simulink model "r2_b8a4x128f_4gbe"  (R2012b)
(part 4 of 182)

      |     current_names = textscan(strtrim(strrep(strrep(get_param(blk, 'names'), ']', ''), '[', '')), '%s');
      |     current_names = current_names{1};
      |     numios = length(current_names);
      |     if length(current_widths) ~= numios,
      |         error('%d field names specified, but %d widths?', numios, length(current_widths));
      |     end
      | end
      | total_width = 0;
      | for ctr = 1 : length(current_widths),
      |     total_width = total_width + current_widths(ctr);
      | end
      | if total_width > 32,
      |     error('Total width must be 32 or less, set to %d.', total_width);
      | end
      mask Callback arith_types:
      | blk = gcb;
      | mode = get_param(blk, 'mode');
      | current_types = eval(get_param(blk, 'arith_types'));
      | numios = length(current_types);
      | if (strcmp(mode, 'one value') || strcmp(mode, 'fields of equal size')) && (length(current_types) > 1),
      |     error('Only one type may be specified for this mode.');
      | elseif strcmp(mode, 'fields of arbitrary size')
      |     current_names = textscan(strtrim(strrep(strrep(get_param(blk, 'names'), ']', ''), '[', '')), '%s');
      |     current_names = current_names{1};
      |     numios = length(current_names);
      |     if length(current_types) ~= numios,
      |         error('%d field names specified, but %d types?', numios, length(current_types));
      |     end
      | end
      | problem = 0;
      | for ctr = 1 : numios,
      |     t = current_types(ctr);
      |     if (t < 0) || (t > 2),
      |         problem = t;
      |         ctr = numios + 1;
      |     end
      | end
      | if problem ~= 0,
      |     error('Type cannot be %i, must be 0, 1 or 2.', problem);
      | end
      mask Callback bin_pts:
      | blk = gcb;
      | mode = get_param(blk, 'mode');
      | current_bins = eval(get_param(blk, 'bin_pts'));
      | if (strcmp(mode, 'one value') || strcmp(mode, 'fields of equal size')) && (length(current_bins) > 1),
      |     error('Only one binary pt may be specified for this mode.');
      | elseif strcmp(mode, 'fields of arbitrary size')
      |     current_names = textscan(strtrim(strrep(strrep(get_param(blk, 'names'), ']', ''), '[', '')), '%s');
      |     current_names = current_names{1};
      |     numios = length(current_names);
      |     if length(current_bins) ~= numios,
      |         error('%d field names specified, but %d binary pts?', numios, length(current_bins));
      |     end
      | end
  status1 : Subsystem  Tag=xps:sw_reg  AncestorBlock=xps_library/software register  mask(swreg){mode=fields of equal size, io_dir=To Processor, io_delay=2, sample_period=1, names=[gbe_down rx_dest_err feng_rx_err fft_err feng_qdr_err feng_chk_err adc_over noise_diode_en vacc_err rx_bad_pkt rx_bad_frame tx_over xeng_bad_dat pack_err rxing_data txing_data flushed], bitwidths=1, arith_types=2, bin_pts=0, sim_port=off, show_format=off}
      mask prompts: io_dir "I/O direction"; io_delay "I/O delay"; sample_period "Sample period"; names "Names [msb ... lsb]:"; bitwidths "Bitwidth:"; arith_types "Type (ufix=0, fix=1, bool=2):"; bin_pts "Binary pt:"; sim_port "Provide sim input/output?"; show_format "Print format string?"
      mask init:
      | swreg_init(gcb)
      settings: AttributesFormatString=17 outputs
      mask TypeOptions mode: one value | fields of equal size | fields of arbitrary size
      mask Callback mode: swreg_cb(gcb);
      mask TypeOptions io_dir: To Processor | From Processor
      mask Callback io_dir:
      | mask_enables = get_param(gcb, 'MaskEnables');
      | mask_names = get_param(gcb, 'MaskNames');
      | if strcmp(get_param(gcb, 'io_dir'), 'To Processor'),
      |     mask_enables{ismember(mask_names, 'sample_period')} = 'off';
      | else
      |     mask_enables{ismember(mask_names, 'sample_period')} = 'on';
      | end
      | set_param(gcb, 'MaskEnables', mask_enables);
      mask Callback bitwidths:
      | blk = gcb;
      | mode = get_param(blk, 'mode');
      | current_widths = eval(get_param(blk, 'bitwidths'));
      | if (strcmp(mode, 'one value') || strcmp(mode, 'fields of equal size')) && (length(current_widths) > 1),
      |     error('Only one width may be specified for this mode.');
      | elseif strcmp(mode, 'fields of arbitrary size')
      |     current_names = textscan(strtrim(strrep(strrep(get_param(blk, 'names'), ']', ''), '[', '')), '%s');
      |     current_names = current_names{1};
      |     numios = length(current_names);
      |     if length(current_widths) ~= numios,
      |         error('%d field names specified, but %d widths?', numios, length(current_widths));
      |     end
      | end
      | total_width = 0;
      | for ctr = 1 : length(current_widths),
      |     total_width = total_width + current_widths(ctr);
      | end
      | if total_width > 32,
      |     error('Total width must be 32 or less, set to %d.', total_width);
      | end
      mask Callback arith_types:
      | blk = gcb;
      | mode = get_param(blk, 'mode');
      | current_types = eval(get_param(blk, 'arith_types'));
      | numios = length(current_types);
      | if (strcmp(mode, 'one value') || strcmp(mode, 'fields of equal size')) && (length(current_types) > 1),
      |     error('Only one type may be specified for this mode.');
      | elseif strcmp(mode, 'fields of arbitrary size')
      |     current_names = textscan(strtrim(strrep(strrep(get_param(blk, 'names'), ']', ''), '[', '')), '%s');
      |     current_names = current_names{1};
      |     numios = length(current_names);
      |     if length(current_types) ~= numios,
      |         error('%d field names specified, but %d types?', numios, length(current_types));
      |     end
      | end
      | problem = 0;
      | for ctr = 1 : numios,
      |     t = current_types(ctr);
      |     if (t < 0) || (t > 2),
      |         problem = t;
      |         ctr = numios + 1;
      |     end
      | end
      | if problem ~= 0,
      |     error('Type cannot be %i, must be 0, 1 or 2.', problem);
      | end
      mask Callback bin_pts:
      | blk = gcb;
      | mode = get_param(blk, 'mode');
      | current_bins = eval(get_param(blk, 'bin_pts'));
      | if (strcmp(mode, 'one value') || strcmp(mode, 'fields of equal size')) && (length(current_bins) > 1),
      |     error('Only one binary pt may be specified for this mode.');
      | elseif strcmp(mode, 'fields of arbitrary size')
      |     current_names = textscan(strtrim(strrep(strrep(get_param(blk, 'names'), ']', ''), '[', '')), '%s');
      |     current_names = current_names{1};
      |     numios = length(current_names);
      |     if length(current_bins) ~= numios,
      |         error('%d field names specified, but %d binary pts?', numios, length(current_bins));
      |     end
      | end
  status2 : Subsystem  Tag=xps:sw_reg  AncestorBlock=xps_library/software register  mask(swreg){mode=fields of equal size, io_dir=To Processor, io_delay=2, sample_period=1, names=[gbe_down rx_dest_err feng_rx_err fft_err feng_qdr_err feng_chk_err adc_over noise_diode_en vacc_err rx_bad_pkt rx_bad_frame tx_over xeng_bad_dat pack_err rxing_data txing_data flushed], bitwidths=1, arith_types=2, bin_pts=0, sim_port=off, show_format=off}
      mask prompts: io_dir "I/O direction"; io_delay "I/O delay"; sample_period "Sample period"; names "Names [msb ... lsb]:"; bitwidths "Bitwidth:"; arith_types "Type (ufix=0, fix=1, bool=2):"; bin_pts "Binary pt:"; sim_port "Provide sim input/output?"; show_format "Print format string?"
      mask init:
      | swreg_init(gcb)
      settings: AttributesFormatString=17 outputs
      mask TypeOptions mode: one value | fields of equal size | fields of arbitrary size
      mask Callback mode: swreg_cb(gcb);
      mask TypeOptions io_dir: To Processor | From Processor
      mask Callback io_dir:
      | mask_enables = get_param(gcb, 'MaskEnables');
      | mask_names = get_param(gcb, 'MaskNames');
      | if strcmp(get_param(gcb, 'io_dir'), 'To Processor'),
      |     mask_enables{ismember(mask_names, 'sample_period')} = 'off';
      | else
      |     mask_enables{ismember(mask_names, 'sample_period')} = 'on';
      | end
      | set_param(gcb, 'MaskEnables', mask_enables);
      mask Callback bitwidths:
      | blk = gcb;
      | mode = get_param(blk, 'mode');
      | current_widths = eval(get_param(blk, 'bitwidths'));
      | if (strcmp(mode, 'one value') || strcmp(mode, 'fields of equal size')) && (length(current_widths) > 1),
      |     error('Only one width may be specified for this mode.');
      | elseif strcmp(mode, 'fields of arbitrary size')
      |     current_names = textscan(strtrim(strrep(strrep(get_param(blk, 'names'), ']', ''), '[', '')), '%s');
      |     current_names = current_names{1};
      |     numios = length(current_names);
      |     if length(current_widths) ~= numios,
      |         error('%d field names specified, but %d widths?', numios, length(current_widths));
      |     end
      | end
      | total_width = 0;
      | for ctr = 1 : length(current_widths),
      |     total_width = total_width + current_widths(ctr);
      | end
      | if total_width > 32,
      |     error('Total width must be 32 or less, set to %d.', total_width);
      | end
      mask Callback arith_types:
      | blk = gcb;
      | mode = get_param(blk, 'mode');
      | current_types = eval(get_param(blk, 'arith_types'));
      | numios = length(current_types);
      | if (strcmp(mode, 'one value') || strcmp(mode, 'fields of equal size')) && (length(current_types) > 1),
      |     error('Only one type may be specified for this mode.');
      | elseif strcmp(mode, 'fields of arbitrary size')
      |     current_names = textscan(strtrim(strrep(strrep(get_param(blk, 'names'), ']', ''), '[', '')), '%s');
      |     current_names = current_names{1};
      |     numios = length(current_names);
      |     if length(current_types) ~= numios,
      |         error('%d field names specified, but %d types?', numios, length(current_types));
      |     end
      | end
      | problem = 0;
      | for ctr = 1 : numios,
      |     t = current_types(ctr);
      |     if (t < 0) || (t > 2),
      |         problem = t;
      |         ctr = numios + 1;
      |     end
      | end
      | if problem ~= 0,
      |     error('Type cannot be %i, must be 0, 1 or 2.', problem);
      | end
      mask Callback bin_pts:
      | blk = gcb;
      | mode = get_param(blk, 'mode');
      | current_bins = eval(get_param(blk, 'bin_pts'));
      | if (strcmp(mode, 'one value') || strcmp(mode, 'fields of equal size')) && (length(current_bins) > 1),
      |     error('Only one binary pt may be specified for this mode.');
      | elseif strcmp(mode, 'fields of arbitrary size')
      |     current_names = textscan(strtrim(strrep(strrep(get_param(blk, 'names'), ']', ''), '[', '')), '%s');
      |     current_names = current_names{1};
      |     numios = length(current_names);
      |     if length(current_bins) ~= numios,
      |         error('%d field names specified, but %d binary pts?', numios, length(current_bins));
      |     end
      | end
  status3 : Subsystem  Tag=xps:sw_reg  AncestorBlock=xps_library/software register  mask(swreg){mode=fields of equal size, io_dir=To Processor, io_delay=2, sample_period=1, names=[gbe_down rx_dest_err feng_rx_err fft_err feng_qdr_err feng_chk_err adc_over noise_diode_en vacc_err rx_bad_pkt rx_bad_frame tx_over xeng_bad_dat pack_err rxing_data txing_data flushed], bitwidths=1, arith_types=2, bin_pts=0, sim_port=off, show_format=off}
      mask prompts: io_dir "I/O direction"; io_delay "I/O delay"; sample_period "Sample period"; names "Names [msb ... lsb]:"; bitwidths "Bitwidth:"; arith_types "Type (ufix=0, fix=1, bool=2):"; bin_pts "Binary pt:"; sim_port "Provide sim input/output?"; show_format "Print format string?"
      mask init:
      | swreg_init(gcb)
      settings: AttributesFormatString=17 outputs
      mask TypeOptions mode: one value | fields of equal size | fields of arbitrary size
      mask Callback mode: swreg_cb(gcb);
      mask TypeOptions io_dir: To Processor | From Processor
      mask Callback io_dir:
      | mask_enables = get_param(gcb, 'MaskEnables');
      | mask_names = get_param(gcb, 'MaskNames');
      | if strcmp(get_param(gcb, 'io_dir'), 'To Processor'),
      |     mask_enables{ismember(mask_names, 'sample_period')} = 'off';
      | else
      |     mask_enables{ismember(mask_names, 'sample_period')} = 'on';
      | end
      | set_param(gcb, 'MaskEnables', mask_enables);
      mask Callback bitwidths:
      | blk = gcb;
      | mode = get_param(blk, 'mode');
      | current_widths = eval(get_param(blk, 'bitwidths'));
      | if (strcmp(mode, 'one value') || strcmp(mode, 'fields of equal size')) && (length(current_widths) > 1),
      |     error('Only one width may be specified for this mode.');
      | elseif strcmp(mode, 'fields of arbitrary size')
      |     current_names = textscan(strtrim(strrep(strrep(get_param(blk, 'names'), ']', ''), '[', '')), '%s');
      |     current_names = current_names{1};
      |     numios = length(current_names);
      |     if length(current_widths) ~= numios,
      |         error('%d field names specified, but %d widths?', numios, length(current_widths));
      |     end
      | end
      | total_width = 0;
      | for ctr = 1 : length(current_widths),
      |     total_width = total_width + current_widths(ctr);
      | end
      | if total_width > 32,
      |     error('Total width must be 32 or less, set to %d.', total_width);
      | end
      mask Callback arith_types:
      | blk = gcb;
      | mode = get_param(blk, 'mode');
      | current_types = eval(get_param(blk, 'arith_types'));
      | numios = length(current_types);
      | if (strcmp(mode, 'one value') || strcmp(mode, 'fields of equal size')) && (length(current_types) > 1),
      |     error('Only one type may be specified for this mode.');
      | elseif strcmp(mode, 'fields of arbitrary size')
      |     current_names = textscan(strtrim(strrep(strrep(get_param(blk, 'names'), ']', ''), '[', '')), '%s');
      |     current_names = current_names{1};
      |     numios = length(current_names);
      |     if length(current_types) ~= numios,
      |         error('%d field names specified, but %d types?', numios, length(current_types));
      |     end
      | end
      | problem = 0;
      | for ctr = 1 : numios,
      |     t = current_types(ctr);
      |     if (t < 0) || (t > 2),
      |         problem = t;
      |         ctr = numios + 1;
      |     end
      | end
      | if problem ~= 0,
      |     error('Type cannot be %i, must be 0, 1 or 2.', problem);
      | end
      mask Callback bin_pts:
      | blk = gcb;
      | mode = get_param(blk, 'mode');
      | current_bins = eval(get_param(blk, 'bin_pts'));
      | if (strcmp(mode, 'one value') || strcmp(mode, 'fields of equal size')) && (length(current_bins) > 1),
      |     error('Only one binary pt may be specified for this mode.');
      | elseif strcmp(mode, 'fields of arbitrary size')
      |     current_names = textscan(strtrim(strrep(strrep(get_param(blk, 'names'), ']', ''), '[', '')), '%s');
      |     current_names = current_names{1};
      |     numios = length(current_names);
      |     if length(current_bins) ~= numios,
      |         error('%d field names specified, but %d binary pts?', numios, length(current_bins));
      |     end
      | end
  sys0 : Subsystem  mask{n_bits_channels=fft_stages-1, n_bits_xengs=n_bits_xengs, n_bits_ants=n_ants, n_bits_xengs_per_fpga=2, xeng_id=0}
      mask prompts: n_bits_channels "frequency channels (2^?)"; n_bits_xengs "xengines in system (2^?)"; n_bits_ants "antennas in system (2^?)"; n_bits_xengs_per_fpga "xengs per fpga (2^?)"; xeng_id "xeng offset in this fpga"
      mask Display: text(0.1, 0.5, 'PREPROCESS -> REORDER -> XENG -> VACC -> PACK');
  sys1 : Subsystem  mask{n_bits_channels=fft_stages-1, n_bits_xengs=n_bits_xengs, n_bits_ants=n_ants, n_bits_xengs_per_fpga=2, xeng_id=1}
      mask prompts: n_bits_channels "frequency channels (2^?)"; n_bits_xengs "xengines in system (2^?)"; n_bits_ants "antennas in systems (2^?)"; n_bits_xengs_per_fpga "xengs per fpga (2^?)"; xeng_id "xeng offset in this fpga"
      mask Display: text(0.1, 0.5, 'PREPROCESS -> REORDER -> XENG -> VACC -> PACK');
  sys2 : Subsystem  mask{n_bits_channels=fft_stages-1, n_bits_xengs=n_bits_xengs, n_bits_ants=n_ants, n_bits_xengs_per_fpga=2, xeng_id=2}
      mask prompts: n_bits_channels "frequency channels (2^?)"; n_bits_xengs "xengines in system (2^?)"; n_bits_ants "antennas in systems (2^?)"; n_bits_xengs_per_fpga "xengs per fpga (2^?)"; xeng_id "xeng offset in this fpga"
      mask Display: text(0.1, 0.5, 'PREPROCESS -> REORDER -> XENG -> VACC -> PACK');
  sys3 : Subsystem  mask{n_bits_channels=fft_stages-1, n_bits_xengs=n_bits_xengs, n_bits_ants=n_ants, n_bits_xengs_per_fpga=2, xeng_id=3}
      mask prompts: n_bits_channels "frequency channels (2^?)"; n_bits_xengs "xengines in system (2^?)"; n_bits_ants "antennas in systems (2^?)"; n_bits_xengs_per_fpga "xengs per fpga (2^?)"; xeng_id "xeng offset in this fpga"
      mask Display: text(0.1, 0.5, 'PREPROCESS -> REORDER -> XENG -> VACC -> PACK');
  tvg_control : Subsystem  Tag=xps:sw_reg  AncestorBlock=xps_library/software register  mask(swreg){mode=fields of arbitrary size, io_dir=From Processor, io_delay=0, sample_period=1, names=[xeng vacc], bitwidths=[2 6], arith_types=[0 0], bin_pts=[0 0], sim_port=off, show_format=on}
      mask prompts: io_dir "I/O direction"; io_delay "I/O delay"; sample_period "Sample period"; names "Names [msb ... lsb]:"; bitwidths "Bitwidths [msb ... lsb]:"; arith_types "Types (ufix=0, fix=1, bool=2) [msb ... lsb]:"; bin_pts "Binary pts [msb ... lsb]:"; sim_port "Provide sim input/output?"; show_format "Print format string?"
      mask init:
      | swreg_init(gcb)
      settings: AttributesFormatString=2 inputs:uf2.0,uf6.0,
      mask TypeOptions mode: one value | fields of equal size | fields of arbitrary size
      mask Callback mode: swreg_cb(gcb);
      mask TypeOptions io_dir: To Processor | From Processor
      mask Callback io_dir:
      | mask_enables = get_param(gcb, 'MaskEnables');
      | mask_names = get_param(gcb, 'MaskNames');
      | if strcmp(get_param(gcb, 'io_dir'), 'To Processor'),
      |     mask_enables{ismember(mask_names, 'sample_period')} = 'off';
      | else
      |     mask_enables{ismember(mask_names, 'sample_period')} = 'on';
      | end
      | set_param(gcb, 'MaskEnables', mask_enables);
      mask Callback bitwidths:
      | blk = gcb;
      | mode = get_param(blk, 'mode');
      | current_widths = eval(get_param(blk, 'bitwidths'));
      | if (strcmp(mode, 'one value') || strcmp(mode, 'fields of equal size')) && (length(current_widths) > 1),
      |     error('Only one width may be specified for this mode.');
      | elseif strcmp(mode, 'fields of arbitrary size')
      |     current_names = textscan(strtrim(strrep(strrep(get_param(blk, 'names'), ']', ''), '[', '')), '%s');
      |     current_names = current_names{1};
      |     numios = length(current_names);
      |     if length(current_widths) ~= numios,
      |         error('%d field names specified, but %d widths?', numios, length(current_widths));
      |     end
      | end
      | total_width = 0;
      | for ctr = 1 : length(current_widths),
      |     total_width = total_width + current_widths(ctr);
      | end
      | if total_width > 32,
      |     error('Total width must be 32 or less, set to %d.', total_width);
      | end
      mask Callback arith_types:
      | blk = gcb;
      | mode = get_param(blk, 'mode');
      | current_types = eval(get_param(blk, 'arith_types'));
      | numios = length(current_types);
      | if (strcmp(mode, 'one value') || strcmp(mode, 'fields of equal size')) && (length(current_types) > 1),
      |     error('Only one type may be specified for this mode.');
      | elseif strcmp(mode, 'fields of arbitrary size')
      |     current_names = textscan(strtrim(strrep(strrep(get_param(blk, 'names'), ']', ''), '[', '')), '%s');
      |     current_names = current_names{1};
      |     numios = length(current_names);
      |     if length(current_types) ~= numios,
      |         error('%d field names specified, but %d types?', numios, length(current_types));
      |     end
      | end
      | problem = 0;
      | for ctr = 1 : numios,
      |     t = current_types(ctr);
      |     if (t < 0) || (t > 2),
      |         problem = t;
      |         ctr = numios + 1;
      |     end
      | end
      | if problem ~= 0,
      |     error('Type cannot be %i, must be 0, 1 or 2.', problem);
      | end
      mask Callback bin_pts:
      | blk = gcb;
      | mode = get_param(blk, 'mode');
      | current_bins = eval(get_param(blk, 'bin_pts'));
      | if (strcmp(mode, 'one value') || strcmp(mode, 'fields of equal size')) && (length(current_bins) > 1),
      |     error('Only one binary pt may be specified for this mode.');
      | elseif strcmp(mode, 'fields of arbitrary size')
      |     current_names = textscan(strtrim(strrep(strrep(get_param(blk, 'names'), ']', ''), '[', '')), '%s');
      |     current_names = current_names{1};
      |     numios = length(current_names);
      |     if length(current_bins) ~= numios,
      |         error('%d field names specified, but %d binary pts?', numios, length(current_bins));
      |     end
      | end
  vacc_errors0 : Subsystem  Tag=xps:sw_reg  AncestorBlock=xps_library/software register  mask(swreg){mode=fields of arbitrary size, io_dir=To Processor, io_delay=1, sample_period=1, names=[calfail inputof rst outputof parity], bitwidths=[6 6 6 6 6], arith_types=[0 0 0 0 0], bin_pts=[0 0 0 0 0], sim_port=off, show_format=on}
      mask prompts: io_dir "I/O direction"; io_delay "I/O delay"; sample_period "Sample period"; names "Names [msb ... lsb]:"; bitwidths "Bitwidths [msb ... lsb]:"; arith_types "Types (ufix=0, fix=1, bool=2) [msb ... lsb]:"; bin_pts "Binary pts [msb ... lsb]:"; sim_port "Provide sim input/output?"; show_format "Print format string?"
      mask init:
      | swreg_init(gcb)
      settings: AttributesFormatString=5 outputs:uf6.0,uf6.0,uf6.0,uf6.0,uf6.0,
      mask TypeOptions mode: one value | fields of equal size | fields of arbitrary size
      mask Callback mode: swreg_cb(gcb);
      mask TypeOptions io_dir: To Processor | From Processor
      mask Callback io_dir:
      | mask_enables = get_param(gcb, 'MaskEnables');
      | mask_names = get_param(gcb, 'MaskNames');
      | if strcmp(get_param(gcb, 'io_dir'), 'To Processor'),
      |     mask_enables{ismember(mask_names, 'sample_period')} = 'off';
      | else
      |     mask_enables{ismember(mask_names, 'sample_period')} = 'on';
      | end
      | set_param(gcb, 'MaskEnables', mask_enables);
      mask Callback bitwidths:
      | blk = gcb;
      | mode = get_param(blk, 'mode');
      | current_widths = eval(get_param(blk, 'bitwidths'));
      | if (strcmp(mode, 'one value') || strcmp(mode, 'fields of equal size')) && (length(current_widths) > 1),
      |     error('Only one width may be specified for this mode.');
      | elseif strcmp(mode, 'fields of arbitrary size')
      |     current_names = textscan(strtrim(strrep(strrep(get_param(blk, 'names'), ']', ''), '[', '')), '%s');
      |     current_names = current_names{1};
      |     numios = length(current_names);
      |     if length(current_widths) ~= numios,
      |         error('%d field names specified, but %d widths?', numios, length(current_widths));
      |     end
      | end
      | total_width = 0;
      | for ctr = 1 : length(current_widths),
      |     total_width = total_width + current_widths(ctr);
      | end
      | if total_width > 32,
      |     error('Total width must be 32 or less, set to %d.', total_width);
      | end
      mask Callback arith_types:
      | blk = gcb;
      | mode = get_param(blk, 'mode');
      | current_types = eval(get_param(blk, 'arith_types'));
      | numios = length(current_types);
      | if (strcmp(mode, 'one value') || strcmp(mode, 'fields of equal size')) && (length(current_types) > 1),
      |     error('Only one type may be specified for this mode.');
      | elseif strcmp(mode, 'fields of arbitrary size')
      |     current_names = textscan(strtrim(strrep(strrep(get_param(blk, 'names'), ']', ''), '[', '')), '%s');
      |     current_names = current_names{1};
      |     numios = length(current_names);
      |     if length(current_types) ~= numios,
      |         error('%d field names specified, but %d types?', numios, length(current_types));
      |     end
      | end
      | problem = 0;
      | for ctr = 1 : numios,
      |     t = current_types(ctr);
      |     if (t < 0) || (t > 2),
      |         problem = t;
      |         ctr = numios + 1;
      |     end
      | end
      | if problem ~= 0,
      |     error('Type cannot be %i, must be 0, 1 or 2.', problem);
      | end
      mask Callback bin_pts:
      | blk = gcb;
      | mode = get_param(blk, 'mode');
      | current_bins = eval(get_param(blk, 'bin_pts'));
      | if (strcmp(mode, 'one value') || strcmp(mode, 'fields of equal size')) && (length(current_bins) > 1),
      |     error('Only one binary pt may be specified for this mode.');
      | elseif strcmp(mode, 'fields of arbitrary size')
      |     current_names = textscan(strtrim(strrep(strrep(get_param(blk, 'names'), ']', ''), '[', '')), '%s');
      |     current_names = current_names{1};
      |     numios = length(current_names);
      |     if length(current_bins) ~= numios,
      |         error('%d field names specified, but %d binary pts?', numios, length(current_bins));
      |     end
      | end
  vacc_errors1 : Subsystem  Tag=xps:sw_reg  AncestorBlock=xps_library/software register  mask(swreg){mode=fields of arbitrary size, io_dir=To Processor, io_delay=0, sample_period=1, names=[calfail inputof rst outputof parity], bitwidths=[6 6 6 6 6], arith_types=[0 0 0 0 0], bin_pts=[0 0 0 0 0], sim_port=off, show_format=on}
      mask prompts: io_dir "I/O direction"; io_delay "I/O delay"; sample_period "Sample period"; names "Names [msb ... lsb]:"; bitwidths "Bitwidths [msb ... lsb]:"; arith_types "Types (ufix=0, fix=1, bool=2) [msb ... lsb]:"; bin_pts "Binary pts [msb ... lsb]:"; sim_port "Provide sim input/output?"; show_format "Print format string?"
      mask init:
      | swreg_init(gcb)
      settings: AttributesFormatString=5 outputs:uf6.0,uf6.0,uf6.0,uf6.0,uf6.0,
      mask TypeOptions mode: one value | fields of equal size | fields of arbitrary size
      mask Callback mode: swreg_cb(gcb);
      mask TypeOptions io_dir: To Processor | From Processor
      mask Callback io_dir:
      | mask_enables = get_param(gcb, 'MaskEnables');
      | mask_names = get_param(gcb, 'MaskNames');
      | if strcmp(get_param(gcb, 'io_dir'), 'To Processor'),
      |     mask_enables{ismember(mask_names, 'sample_period')} = 'off';
      | else
      |     mask_enables{ismember(mask_names, 'sample_period')} = 'on';
      | end
      | set_param(gcb, 'MaskEnables', mask_enables);
      mask Callback bitwidths:
      | blk = gcb;
      | mode = get_param(blk, 'mode');
      | current_widths = eval(get_param(blk, 'bitwidths'));
      | if (strcmp(mode, 'one value') || strcmp(mode, 'fields of equal size')) && (length(current_widths) > 1),
      |     error('Only one width may be specified for this mode.');
      | elseif strcmp(mode, 'fields of arbitrary size')
      |     current_names = textscan(strtrim(strrep(strrep(get_param(blk, 'names'), ']', ''), '[', '')), '%s');
      |     current_names = current_names{1};
      |     numios = length(current_names);
      |     if length(current_widths) ~= numios,
      |         error('%d field names specified, but %d widths?', numios, length(current_widths));
      |     end
      | end
      | total_width = 0;
      | for ctr = 1 : length(current_widths),
      |     total_width = total_width + current_widths(ctr);
      | end
      | if total_width > 32,
      |     error('Total width must be 32 or less, set to %d.', total_width);
      | end
      mask Callback arith_types:
      | blk = gcb;
      | mode = get_param(blk, 'mode');
      | current_types = eval(get_param(blk, 'arith_types'));
      | numios = length(current_types);
      | if (strcmp(mode, 'one value') || strcmp(mode, 'fields of equal size')) && (length(current_types) > 1),
      |     error('Only one type may be specified for this mode.');
      | elseif strcmp(mode, 'fields of arbitrary size')
      |     current_names = textscan(strtrim(strrep(strrep(get_param(blk, 'names'), ']', ''), '[', '')), '%s');
      |     current_names = current_names{1};
      |     numios = length(current_names);
      |     if length(current_types) ~= numios,
      |         error('%d field names specified, but %d types?', numios, length(current_types));
      |     end
      | end
      | problem = 0;
      | for ctr = 1 : numios,
      |     t = current_types(ctr);
      |     if (t < 0) || (t > 2),
      |         problem = t;
      |         ctr = numios + 1;
      |     end
      | end
      | if problem ~= 0,
      |     error('Type cannot be %i, must be 0, 1 or 2.', problem);
      | end
      mask Callback bin_pts:
      | blk = gcb;
      | mode = get_param(blk, 'mode');
      | current_bins = eval(get_param(blk, 'bin_pts'));
      | if (strcmp(mode, 'one value') || strcmp(mode, 'fields of equal size')) && (length(current_bins) > 1),
      |     error('Only one binary pt may be specified for this mode.');
      | elseif strcmp(mode, 'fields of arbitrary size')
      |     current_names = textscan(strtrim(strrep(strrep(get_param(blk, 'names'), ']', ''), '[', '')), '%s');
      |     current_names = current_names{1};
      |     numios = length(current_names);
      |     if length(current_bins) ~= numios,
      |         error('%d field names specified, but %d binary pts?', numios, length(current_bins));
      |     end
      | end
  vacc_errors2 : Subsystem  Tag=xps:sw_reg  AncestorBlock=xps_library/software register  mask(swreg){mode=fields of arbitrary size, io_dir=To Processor, io_delay=0, sample_period=1, names=[calfail inputof rst outputof parity], bitwidths=[6 6 6 6 6], arith_types=[0 0 0 0 0], bin_pts=[0 0 0 0 0], sim_port=off, show_format=on}
      mask prompts: io_dir "I/O direction"; io_delay "I/O delay"; sample_period "Sample period"; names "Names [msb ... lsb]:"; bitwidths "Bitwidths [msb ... lsb]:"; arith_types "Types (ufix=0, fix=1, bool=2) [msb ... lsb]:"; bin_pts "Binary pts [msb ... lsb]:"; sim_port "Provide sim input/output?"; show_format "Print format string?"
      mask init:
      | swreg_init(gcb)
      settings: AttributesFormatString=5 outputs:uf6.0,uf6.0,uf6.0,uf6.0,uf6.0,
      mask TypeOptions mode: one value | fields of equal size | fields of arbitrary size
      mask Callback mode: swreg_cb(gcb);
      mask TypeOptions io_dir: To Processor | From Processor
      mask Callback io_dir:
      | mask_enables = get_param(gcb, 'MaskEnables');
      | mask_names = get_param(gcb, 'MaskNames');
      | if strcmp(get_param(gcb, 'io_dir'), 'To Processor'),
      |     mask_enables{ismember(mask_names, 'sample_period')} = 'off';
      | else
      |     mask_enables{ismember(mask_names, 'sample_period')} = 'on';
      | end
      | set_param(gcb, 'MaskEnables', mask_enables);
      mask Callback bitwidths:
      | blk = gcb;
      | mode = get_param(blk, 'mode');
      | current_widths = eval(get_param(blk, 'bitwidths'));
      | if (strcmp(mode, 'one value') || strcmp(mode, 'fields of equal size')) && (length(current_widths) > 1),
      |     error('Only one width may be specified for this mode.');
      | elseif strcmp(mode, 'fields of arbitrary size')
      |     current_names = textscan(strtrim(strrep(strrep(get_param(blk, 'names'), ']', ''), '[', '')), '%s');
      |     current_names = current_names{1};
      |     numios = length(current_names);
      |     if length(current_widths) ~= numios,
      |         error('%d field names specified, but %d widths?', numios, length(current_widths));
      |     end
      | end
      | total_width = 0;
      | for ctr = 1 : length(current_widths),
      |     total_width = total_width + current_widths(ctr);
      | end
      | if total_width > 32,
      |     error('Total width must be 32 or less, set to %d.', total_width);
      | end
      mask Callback arith_types:
      | blk = gcb;
      | mode = get_param(blk, 'mode');
      | current_types = eval(get_param(blk, 'arith_types'));
      | numios = length(current_types);
      | if (strcmp(mode, 'one value') || strcmp(mode, 'fields of equal size')) && (length(current_types) > 1),
      |     error('Only one type may be specified for this mode.');
      | elseif strcmp(mode, 'fields of arbitrary size')
      |     current_names = textscan(strtrim(strrep(strrep(get_param(blk, 'names'), ']', ''), '[', '')), '%s');
      |     current_names = current_names{1};
      |     numios = length(current_names);
      |     if length(current_types) ~= numios,
      |         error('%d field names specified, but %d types?', numios, length(current_types));
      |     end
      | end
      | problem = 0;
      | for ctr = 1 : numios,
      |     t = current_types(ctr);
      |     if (t < 0) || (t > 2),
      |         problem = t;
      |         ctr = numios + 1;
      |     end
      | end
      | if problem ~= 0,
      |     error('Type cannot be %i, must be 0, 1 or 2.', problem);
      | end
      mask Callback bin_pts:
      | blk = gcb;
      | mode = get_param(blk, 'mode');
      | current_bins = eval(get_param(blk, 'bin_pts'));
      | if (strcmp(mode, 'one value') || strcmp(mode, 'fields of equal size')) && (length(current_bins) > 1),
      |     error('Only one binary pt may be specified for this mode.');
      | elseif strcmp(mode, 'fields of arbitrary size')
      |     current_names = textscan(strtrim(strrep(strrep(get_param(blk, 'names'), ']', ''), '[', '')), '%s');
      |     current_names = current_names{1};
      |     numios = length(current_names);
      |     if length(current_bins) ~= numios,
      |         error('%d field names specified, but %d binary pts?', numios, length(current_bins));
      |     end
      | end
  vacc_errors3 : Subsystem  Tag=xps:sw_reg  AncestorBlock=xps_library/software register  mask(swreg){mode=fields of arbitrary size, io_dir=To Processor, io_delay=1, sample_period=1, names=[calfail inputof rst outputof parity], bitwidths=[6 6 6 6 6], arith_types=[0 0 0 0 0], bin_pts=[0 0 0 0 0], sim_port=off, show_format=on}
      mask prompts: io_dir "I/O direction"; io_delay "I/O delay"; sample_period "Sample period"; names "Names [msb ... lsb]:"; bitwidths "Bitwidths [msb ... lsb]:"; arith_types "Types (ufix=0, fix=1, bool=2) [msb ... lsb]:"; bin_pts "Binary pts [msb ... lsb]:"; sim_port "Provide sim input/output?"; show_format "Print format string?"
      mask init:
      | swreg_init(gcb)
      settings: AttributesFormatString=5 outputs:uf6.0,uf6.0,uf6.0,uf6.0,uf6.0,
      mask TypeOptions mode: one value | fields of equal size | fields of arbitrary size
      mask Callback mode: swreg_cb(gcb);
      mask TypeOptions io_dir: To Processor | From Processor
      mask Callback io_dir:
      | mask_enables = get_param(gcb, 'MaskEnables');
      | mask_names = get_param(gcb, 'MaskNames');
      | if strcmp(get_param(gcb, 'io_dir'), 'To Processor'),
      |     mask_enables{ismember(mask_names, 'sample_period')} = 'off';
      | else
      |     mask_enables{ismember(mask_names, 'sample_period')} = 'on';
      | end
      | set_param(gcb, 'MaskEnables', mask_enables);
      mask Callback bitwidths:
      | blk = gcb;
      | mode = get_param(blk, 'mode');
      | current_widths = eval(get_param(blk, 'bitwidths'));
      | if (strcmp(mode, 'one value') || strcmp(mode, 'fields of equal size')) && (length(current_widths) > 1),
      |     error('Only one width may be specified for this mode.');
      | elseif strcmp(mode, 'fields of arbitrary size')
      |     current_names = textscan(strtrim(strrep(strrep(get_param(blk, 'names'), ']', ''), '[', '')), '%s');
      |     current_names = current_names{1};
      |     numios = length(current_names);
      |     if length(current_widths) ~= numios,
      |         error('%d field names specified, but %d widths?', numios, length(current_widths));
      |     end
      | end
      | total_width = 0;
      | for ctr = 1 : length(current_widths),
      |     total_width = total_width + current_widths(ctr);
      | end
      | if total_width > 32,
      |     error('Total width must be 32 or less, set to %d.', total_width);
      | end
      mask Callback arith_types:
      | blk = gcb;
      | mode = get_param(blk, 'mode');
      | current_types = eval(get_param(blk, 'arith_types'));
      | numios = length(current_types);
      | if (strcmp(mode, 'one value') || strcmp(mode, 'fields of equal size')) && (length(current_types) > 1),
      |     error('Only one type may be specified for this mode.');
      | elseif strcmp(mode, 'fields of arbitrary size')
      |     current_names = textscan(strtrim(strrep(strrep(get_param(blk, 'names'), ']', ''), '[', '')), '%s');
      |     current_names = current_names{1};
      |     numios = length(current_names);
      |     if length(current_types) ~= numios,
      |         error('%d field names specified, but %d types?', numios, length(current_types));
      |     end
      | end
      | problem = 0;
      | for ctr = 1 : numios,
      |     t = current_types(ctr);
      |     if (t < 0) || (t > 2),
      |         problem = t;
      |         ctr = numios + 1;
      |     end
      | end
      | if problem ~= 0,
      |     error('Type cannot be %i, must be 0, 1 or 2.', problem);
      | end
      mask Callback bin_pts:
      | blk = gcb;
      | mode = get_param(blk, 'mode');
      | current_bins = eval(get_param(blk, 'bin_pts'));
      | if (strcmp(mode, 'one value') || strcmp(mode, 'fields of equal size')) && (length(current_bins) > 1),
      |     error('Only one binary pt may be specified for this mode.');
      | elseif strcmp(mode, 'fields of arbitrary size')
      |     current_names = textscan(strtrim(strrep(strrep(get_param(blk, 'names'), ']', ''), '[', '')), '%s');
      |     current_names = current_names{1};
      |     numios = length(current_names);
      |     if length(current_bins) ~= numios,
      |         error('%d field names specified, but %d binary pts?', numios, length(current_bins));
      |     end
      | end
  vacc_ld_status0 : Subsystem  Tag=xps:sw_reg  AncestorBlock=xps_library/software register  mask(swreg){mode=fields of equal size, io_dir=To Processor, io_delay=1, sample_period=1, names=[armcnt ldcnt], bitwidths=16, arith_types=0, bin_pts=0, sim_port=off, show_format=on}
      mask prompts: io_dir "I/O direction"; io_delay "I/O delay"; sample_period "Sample period"; names "Names [msb ... lsb]:"; bitwidths "Bitwidth:"; arith_types "Type (ufix=0, fix=1, bool=2):"; bin_pts "Binary pt:"; sim_port "Provide sim input/output?"; show_format "Print format string?"
      mask init:
      | swreg_init(gcb)
      settings: AttributesFormatString=2 outputs:uf16.0,uf16.0,
      mask TypeOptions mode: one value | fields of equal size | fields of arbitrary size
      mask Callback mode: swreg_cb(gcb);
      mask TypeOptions io_dir: To Processor | From Processor
      mask Callback io_dir:
      | mask_enables = get_param(gcb, 'MaskEnables');
      | mask_names = get_param(gcb, 'MaskNames');
      | if strcmp(get_param(gcb, 'io_dir'), 'To Processor'),
      |     mask_enables{ismember(mask_names, 'sample_period')} = 'off';
      | else
      |     mask_enables{ismember(mask_names, 'sample_period')} = 'on';
      | end
      | set_param(gcb, 'MaskEnables', mask_enables);
      mask Callback bitwidths:
      | blk = gcb;
      | mode = get_param(blk, 'mode');
      | current_widths = eval(get_param(blk, 'bitwidths'));
      | if (strcmp(mode, 'one value') || strcmp(mode, 'fields of equal size')) && (length(current_widths) > 1),
      |     error('Only one width may be specified for this mode.');
      | elseif strcmp(mode, 'fields of arbitrary size')
      |     current_names = textscan(strtrim(strrep(strrep(get_param(blk, 'names'), ']', ''), '[', '')), '%s');
      |     current_names = current_names{1};
      |     numios = length(current_names);
      |     if length(current_widths) ~= numios,
      |         error('%d field names specified, but %d widths?', numios, length(current_widths));
      |     end
      | end
      | total_width = 0;
      | for ctr = 1 : length(current_widths),
      |     total_width = total_width + current_widths(ctr);
      | end
      | if total_width > 32,
      |     error('Total width must be 32 or less, set to %d.', total_width);
      | end
      mask Callback arith_types:
      | blk = gcb;
      | mode = get_param(blk, 'mode');
      | current_types = eval(get_param(blk, 'arith_types'));
      | numios = length(current_types);
      | if (strcmp(mode, 'one value') || strcmp(mode, 'fields of equal size')) && (length(current_types) > 1),
      |     error('Only one type may be specified for this mode.');
      | elseif strcmp(mode, 'fields of arbitrary size')
      |     current_names = textscan(strtrim(strrep(strrep(get_param(blk, 'names'), ']', ''), '[', '')), '%s');
      |     current_names = current_names{1};
      |     numios = length(current_names);
      |     if length(current_types) ~= numios,
      |         error('%d field names specified, but %d types?', numios, length(current_types));
      |     end
      | end
      | problem = 0;
      | for ctr = 1 : numios,
      |     t = current_types(ctr);
      |     if (t < 0) || (t > 2),
      |         problem = t;
      |         ctr = numios + 1;
      |     end
      | end
      | if problem ~= 0,
      |     error('Type cannot be %i, must be 0, 1 or 2.', problem);
      | end
      mask Callback bin_pts:
      | blk = gcb;
      | mode = get_param(blk, 'mode');
      | current_bins = eval(get_param(blk, 'bin_pts'));
      | if (strcmp(mode, 'one value') || strcmp(mode, 'fields of equal size')) && (length(current_bins) > 1),
      |     error('Only one binary pt may be specified for this mode.');
      | elseif strcmp(mode, 'fields of arbitrary size')
      |     current_names = textscan(strtrim(strrep(strrep(get_param(blk, 'names'), ']', ''), '[', '')), '%s');
      |     current_names = current_names{1};
      |     numios = length(current_names);
      |     if length(current_bins) ~= numios,
      |         error('%d field names specified, but %d binary pts?', numios, length(current_bins));
      |     end
      | end
  vacc_ld_status1 : Subsystem  Tag=xps:sw_reg  AncestorBlock=xps_library/software register  mask(swreg){mode=fields of equal size, io_dir=To Processor, io_delay=0, sample_period=1, names=[armcnt ldcnt], bitwidths=16, arith_types=0, bin_pts=0, sim_port=off, show_format=on}
      mask prompts: io_dir "I/O direction"; io_delay "I/O delay"; sample_period "Sample period"; names "Names [msb ... lsb]:"; bitwidths "Bitwidth:"; arith_types "Type (ufix=0, fix=1, bool=2):"; bin_pts "Binary pt:"; sim_port "Provide sim input/output?"; show_format "Print format string?"
      mask init:
      | swreg_init(gcb)
      settings: AttributesFormatString=2 outputs:uf16.0,uf16.0,
      mask TypeOptions mode: one value | fields of equal size | fields of arbitrary size
      mask Callback mode: swreg_cb(gcb);
      mask TypeOptions io_dir: To Processor | From Processor
      mask Callback io_dir:
      | mask_enables = get_param(gcb, 'MaskEnables');
      | mask_names = get_param(gcb, 'MaskNames');
      | if strcmp(get_param(gcb, 'io_dir'), 'To Processor'),
      |     mask_enables{ismember(mask_names, 'sample_period')} = 'off';
      | else
      |     mask_enables{ismember(mask_names, 'sample_period')} = 'on';
      | end
      | set_param(gcb, 'MaskEnables', mask_enables);
      mask Callback bitwidths:
      | blk = gcb;
      | mode = get_param(blk, 'mode');
      | current_widths = eval(get_param(blk, 'bitwidths'));
      | if (strcmp(mode, 'one value') || strcmp(mode, 'fields of equal size')) && (length(current_widths) > 1),
      |     error('Only one width may be specified for this mode.');
      | elseif strcmp(mode, 'fields of arbitrary size')
      |     current_names = textscan(strtrim(strrep(strrep(get_param(blk, 'names'), ']', ''), '[', '')), '%s');
      |     current_names = current_names{1};
      |     numios = length(current_names);
      |     if length(current_widths) ~= numios,
      |         error('%d field names specified, but %d widths?', numios, length(current_widths));
      |     end
      | end
      | total_width = 0;
      | for ctr = 1 : length(current_widths),
      |     total_width = total_width + current_widths(ctr);
      | end
      | if total_width > 32,
      |     error('Total width must be 32 or less, set to %d.', total_width);
      | end
      mask Callback arith_types:
      | blk = gcb;
      | mode = get_param(blk, 'mode');
      | current_types = eval(get_param(blk, 'arith_types'));
      | numios = length(current_types);
      | if (strcmp(mode, 'one value') || strcmp(mode, 'fields of equal size')) && (length(current_types) > 1),
      |     error('Only one type may be specified for this mode.');
      | elseif strcmp(mode, 'fields of arbitrary size')
      |     current_names = textscan(strtrim(strrep(strrep(get_param(blk, 'names'), ']', ''), '[', '')), '%s');
      |     current_names = current_names{1};
      |     numios = length(current_names);
      |     if length(current_types) ~= numios,
      |         error('%d field names specified, but %d types?', numios, length(current_types));
      |     end
      | end
      | problem = 0;
      | for ctr = 1 : numios,
      |     t = current_types(ctr);
      |     if (t < 0) || (t > 2),
      |         problem = t;
      |         ctr = numios + 1;
      |     end
      | end
      | if problem ~= 0,
      |     error('Type cannot be %i, must be 0, 1 or 2.', problem);
      | end
      mask Callback bin_pts:
      | blk = gcb;
      | mode = get_param(blk, 'mode');
      | current_bins = eval(get_param(blk, 'bin_pts'));
      | if (strcmp(mode, 'one value') || strcmp(mode, 'fields of equal size')) && (length(current_bins) > 1),
      |     error('Only one binary pt may be specified for this mode.');
      | elseif strcmp(mode, 'fields of arbitrary size')
      |     current_names = textscan(strtrim(strrep(strrep(get_param(blk, 'names'), ']', ''), '[', '')), '%s');
      |     current_names = current_names{1};
      |     numios = length(current_names);
      |     if length(current_bins) ~= numios,
      |         error('%d field names specified, but %d binary pts?', numios, length(current_bins));
      |     end
      | end
  vacc_ld_status2 : Subsystem  Tag=xps:sw_reg  AncestorBlock=xps_library/software register  mask(swreg){mode=fields of equal size, io_dir=To Processor, io_delay=1, sample_period=1, names=[armcnt ldcnt], bitwidths=16, arith_types=0, bin_pts=0, sim_port=off, show_format=on}
      mask prompts: io_dir "I/O direction"; io_delay "I/O delay"; sample_period "Sample period"; names "Names [msb ... lsb]:"; bitwidths "Bitwidth:"; arith_types "Type (ufix=0, fix=1, bool=2):"; bin_pts "Binary pt:"; sim_port "Provide sim input/output?"; show_format "Print format string?"
      mask init:
      | swreg_init(gcb)
      settings: AttributesFormatString=2 outputs:uf16.0,uf16.0,
      mask TypeOptions mode: one value | fields of equal size | fields of arbitrary size
      mask Callback mode: swreg_cb(gcb);
      mask TypeOptions io_dir: To Processor | From Processor
      mask Callback io_dir:
      | mask_enables = get_param(gcb, 'MaskEnables');
      | mask_names = get_param(gcb, 'MaskNames');
      | if strcmp(get_param(gcb, 'io_dir'), 'To Processor'),
      |     mask_enables{ismember(mask_names, 'sample_period')} = 'off';
      | else
      |     mask_enables{ismember(mask_names, 'sample_period')} = 'on';
      | end
      | set_param(gcb, 'MaskEnables', mask_enables);
      mask Callback bitwidths:
      | blk = gcb;
      | mode = get_param(blk, 'mode');
      | current_widths = eval(get_param(blk, 'bitwidths'));
      | if (strcmp(mode, 'one value') || strcmp(mode, 'fields of equal size')) && (length(current_widths) > 1),
      |     error('Only one width may be specified for this mode.');
      | elseif strcmp(mode, 'fields of arbitrary size')
      |     current_names = textscan(strtrim(strrep(strrep(get_param(blk, 'names'), ']', ''), '[', '')), '%s');
      |     current_names = current_names{1};
      |     numios = length(current_names);
      |     if length(current_widths) ~= numios,
      |         error('%d field names specified, but %d widths?', numios, length(current_widths));
      |     end
      | end
      | total_width = 0;
      | for ctr = 1 : length(current_widths),
      |     total_width = total_width + current_widths(ctr);
      | end
      | if total_width > 32,
      |     error('Total width must be 32 or less, set to %d.', total_width);
      | end
      mask Callback arith_types:
      | blk = gcb;
      | mode = get_param(blk, 'mode');
      | current_types = eval(get_param(blk, 'arith_types'));
      | numios = length(current_types);
      | if (strcmp(mode, 'one value') || strcmp(mode, 'fields of equal size')) && (length(current_types) > 1),
      |     error('Only one type may be specified for this mode.');
      | elseif strcmp(mode, 'fields of arbitrary size')
      |     current_names = textscan(strtrim(strrep(strrep(get_param(blk, 'names'), ']', ''), '[', '')), '%s');
      |     current_names = current_names{1};
      |     numios = length(current_names);
      |     if length(current_types) ~= numios,
      |         error('%d field names specified, but %d types?', numios, length(current_types));
      |     end
      | end
      | problem = 0;
      | for ctr = 1 : numios,
      |     t = current_types(ctr);
      |     if (t < 0) || (t > 2),
      |         problem = t;
      |         ctr = numios + 1;
      |     end
      | end
      | if problem ~= 0,
      |     error('Type cannot be %i, must be 0, 1 or 2.', problem);
      | end
      mask Callback bin_pts:
      | blk = gcb;
      | mode = get_param(blk, 'mode');
      | current_bins = eval(get_param(blk, 'bin_pts'));
      | if (strcmp(mode, 'one value') || strcmp(mode, 'fields of equal size')) && (length(current_bins) > 1),
      |     error('Only one binary pt may be specified for this mode.');
      | elseif strcmp(mode, 'fields of arbitrary size')
      |     current_names = textscan(strtrim(strrep(strrep(get_param(blk, 'names'), ']', ''), '[', '')), '%s');
      |     current_names = current_names{1};
      |     numios = length(current_names);
      |     if length(current_bins) ~= numios,
      |         error('%d field names specified, but %d binary pts?', numios, length(current_bins));
      |     end
      | end
  vacc_ld_status3 : Subsystem  Tag=xps:sw_reg  AncestorBlock=xps_library/software register  mask(swreg){mode=fields of equal size, io_dir=To Processor, io_delay=1, sample_period=1, names=[armcnt ldcnt], bitwidths=16, arith_types=0, bin_pts=0, sim_port=off, show_format=on}
      mask prompts: io_dir "I/O direction"; io_delay "I/O delay"; sample_period "Sample period"; names "Names [msb ... lsb]:"; bitwidths "Bitwidth:"; arith_types "Type (ufix=0, fix=1, bool=2):"; bin_pts "Binary pt:"; sim_port "Provide sim input/output?"; show_format "Print format string?"
      mask init:
      | swreg_init(gcb)
      settings: AttributesFormatString=2 outputs:uf16.0,uf16.0,
      mask TypeOptions mode: one value | fields of equal size | fields of arbitrary size
      mask Callback mode: swreg_cb(gcb);
      mask TypeOptions io_dir: To Processor | From Processor
      mask Callback io_dir:
      | mask_enables = get_param(gcb, 'MaskEnables');
      | mask_names = get_param(gcb, 'MaskNames');
      | if strcmp(get_param(gcb, 'io_dir'), 'To Processor'),
      |     mask_enables{ismember(mask_names, 'sample_period')} = 'off';
      | else
      |     mask_enables{ismember(mask_names, 'sample_period')} = 'on';
      | end
      | set_param(gcb, 'MaskEnables', mask_enables);
      mask Callback bitwidths:
      | blk = gcb;
      | mode = get_param(blk, 'mode');
      | current_widths = eval(get_param(blk, 'bitwidths'));
      | if (strcmp(mode, 'one value') || strcmp(mode, 'fields of equal size')) && (length(current_widths) > 1),
      |     error('Only one width may be specified for this mode.');
      | elseif strcmp(mode, 'fields of arbitrary size')
      |     current_names = textscan(strtrim(strrep(strrep(get_param(blk, 'names'), ']', ''), '[', '')), '%s');
      |     current_names = current_names{1};
      |     numios = length(current_names);
      |     if length(current_widths) ~= numios,
      |         error('%d field names specified, but %d widths?', numios, length(current_widths));
      |     end
      | end
      | total_width = 0;
      | for ctr = 1 : length(current_widths),
      |     total_width = total_width + current_widths(ctr);
      | end
      | if total_width > 32,
      |     error('Total width must be 32 or less, set to %d.', total_width);
      | end
      mask Callback arith_types:
      | blk = gcb;
      | mode = get_param(blk, 'mode');
      | current_types = eval(get_param(blk, 'arith_types'));
      | numios = length(current_types);
      | if (strcmp(mode, 'one value') || strcmp(mode, 'fields of equal size')) && (length(current_types) > 1),
      |     error('Only one type may be specified for this mode.');
      | elseif strcmp(mode, 'fields of arbitrary size')
      |     current_names = textscan(strtrim(strrep(strrep(get_param(blk, 'names'), ']', ''), '[', '')), '%s');
      |     current_names = current_names{1};
      |     numios = length(current_names);
      |     if length(current_types) ~= numios,
      |         error('%d field names specified, but %d types?', numios, length(current_types));
      |     end
      | end
      | problem = 0;
      | for ctr = 1 : numios,
      |     t = current_types(ctr);
      |     if (t < 0) || (t > 2),
      |         problem = t;
      |         ctr = numios + 1;
      |     end
      | end
      | if problem ~= 0,
      |     error('Type cannot be %i, must be 0, 1 or 2.', problem);
      | end
      mask Callback bin_pts:
      | blk = gcb;
      | mode = get_param(blk, 'mode');
      | current_bins = eval(get_param(blk, 'bin_pts'));
      | if (strcmp(mode, 'one value') || strcmp(mode, 'fields of equal size')) && (length(current_bins) > 1),
      |     error('Only one binary pt may be specified for this mode.');
      | elseif strcmp(mode, 'fields of arbitrary size')
      |     current_names = textscan(strtrim(strrep(strrep(get_param(blk, 'names'), ']', ''), '[', '')), '%s');
      |     current_names = current_names{1};
      |     numios = length(current_names);
      |     if length(current_bins) ~= numios,
      |         error('%d field names specified, but %d binary pts?', numios, length(current_bins));
      |     end
      | end
  vacc_monitor1 : Subsystem
  vacc_monitor10 : Subsystem
  vacc_monitor11 : Subsystem
  vacc_monitor12 : Subsystem
  vacc_monitor2 : Subsystem
  vacc_monitor3 : Subsystem
  vacc_monitor4 : Subsystem
  vacc_monitor5 : Subsystem
  vacc_monitor6 : Subsystem
  vacc_monitor7 : Subsystem
  vacc_monitor8 : Subsystem
  vacc_monitor9 : Subsystem
  vacc_time_lsw : Subsystem  Tag=xps:sw_reg  AncestorBlock=xps_library/software register  mask(swreg){mode=one value, io_dir=From Processor, io_delay=0, sample_period=1, names=lsw, bitwidths=32, arith_types=0, bin_pts=0, sim_port=off, show_format=off}
      mask prompts: io_dir "I/O direction"; io_delay "I/O delay"; sample_period "Sample period"; names "Name:"; bitwidths "Bitwidth:"; arith_types "Type (ufix=0, fix=1, bool=2):"; bin_pts "Binary pt:"; sim_port "Provide sim input/output?"; show_format "Print format string?"
      mask init:
      | swreg_init(gcb)
      settings: AttributesFormatString=1input
      mask TypeOptions mode: one value | fields of equal size | fields of arbitrary size
      mask Callback mode: swreg_cb(gcb);
      mask TypeOptions io_dir: To Processor | From Processor
      mask Callback io_dir:
      | mask_enables = get_param(gcb, 'MaskEnables');
      | mask_names = get_param(gcb, 'MaskNames');
      | if strcmp(get_param(gcb, 'io_dir'), 'To Processor'),
      |     mask_enables{ismember(mask_names, 'sample_period')} = 'off';
      | else
      |     mask_enables{ismember(mask_names, 'sample_period')} = 'on';
      | end
      | set_param(gcb, 'MaskEnables', mask_enables);
      mask Callback bitwidths:
      | blk = gcb;
      | mode = get_param(blk, 'mode');
      | current_widths = eval(get_param(blk, 'bitwidths'));
      | if (strcmp(mode, 'one value') || strcmp(mode, 'fields of equal size')) && (length(current_widths) > 1),
      |     error('Only one width may be specified for this mode.');
      | elseif strcmp(mode, 'fields of arbitrary size')
      |     current_names = textscan(strtrim(strrep(strrep(get_param(blk, 'names'), ']', ''), '[', '')), '%s');
      |     current_names = current_names{1};
      |     numios = length(current_names);
      |     if length(current_widths) ~= numios,
      |         error('%d field names specified, but %d widths?', numios, length(current_widths));
      |     end
      | end
      | total_width = 0;
      | for ctr = 1 : length(current_widths),
      |     total_width = total_width + current_widths(ctr);
      | end
      | if total_width > 32,
      |     error('Total width must be 32 or less, set to %d.', total_width);
      | end
      mask Callback arith_types:
      | blk = gcb;
      | mode = get_param(blk, 'mode');
      | current_types = eval(get_param(blk, 'arith_types'));
      | numios = length(current_types);
      | if (strcmp(mode, 'one value') || strcmp(mode, 'fields of equal size')) && (length(current_types) > 1),
      |     error('Only one type may be specified for this mode.');
      | elseif strcmp(mode, 'fields of arbitrary size')
      |     current_names = textscan(strtrim(strrep(strrep(get_param(blk, 'names'), ']', ''), '[', '')), '%s');
      |     current_names = current_names{1};
      |     numios = length(current_names);
      |     if length(current_types) ~= numios,
      |         error('%d field names specified, but %d types?', numios, length(current_types));
      |     end
      | end
      | problem = 0;
      | for ctr = 1 : numios,
      |     t = current_types(ctr);
      |     if (t < 0) || (t > 2),
      |         problem = t;
      |         ctr = numios + 1;
      |     end
      | end
      | if problem ~= 0,
      |     error('Type cannot be %i, must be 0, 1 or 2.', problem);
      | end
      mask Callback bin_pts:
      | blk = gcb;
      | mode = get_param(blk, 'mode');
      | current_bins = eval(get_param(blk, 'bin_pts'));
      | if (strcmp(mode, 'one value') || strcmp(mode, 'fields of equal size')) && (length(current_bins) > 1),
      |     error('Only one binary pt may be specified for this mode.');
      | elseif strcmp(mode, 'fields of arbitrary size')
      |     current_names = textscan(strtrim(strrep(strrep(get_param(blk, 'names'), ']', ''), '[', '')), '%s');
      |     current_names = current_names{1};
      |     numios = length(current_names);
      |     if length(current_bins) ~= numios,
      |         error('%d field names specified, but %d binary pts?', numios, length(current_bins));
      |     end
      | end
  vacc_time_msw : Subsystem  Tag=xps:sw_reg  AncestorBlock=xps_library/software register  mask(swreg){mode=fields of arbitrary size, io_dir=From Processor, io_delay=0, sample_period=1, names=[arm immediate msw], bitwidths=[1 1 16], arith_types=[2 2 0], bin_pts=[0 0 0], sim_port=off, show_format=off}
      mask prompts: io_dir "I/O direction"; io_delay "I/O delay"; sample_period "Sample period"; names "Names [msb ... lsb]:"; bitwidths "Bitwidths [msb ... lsb]:"; arith_types "Types (ufix=0, fix=1, bool=2) [msb ... lsb]:"; bin_pts "Binary pts [msb ... lsb]:"; sim_port "Provide sim input/output?"; show_format "Print format string?"
      mask init:
      | swreg_init(gcb)
      settings: AttributesFormatString=3 inputs
      mask TypeOptions mode: one value | fields of equal size | fields of arbitrary size
      mask Callback mode: swreg_cb(gcb);
      mask TypeOptions io_dir: To Processor | From Processor
      mask Callback io_dir:
      | mask_enables = get_param(gcb, 'MaskEnables');
      | mask_names = get_param(gcb, 'MaskNames');
      | if strcmp(get_param(gcb, 'io_dir'), 'To Processor'),
      |     mask_enables{ismember(mask_names, 'sample_period')} = 'off';
      | else
      |     mask_enables{ismember(mask_names, 'sample_period')} = 'on';
      | end
      | set_param(gcb, 'MaskEnables', mask_enables);
      mask Callback bitwidths:
      | blk = gcb;
      | mode = get_param(blk, 'mode');
      | current_widths = eval(get_param(blk, 'bitwidths'));
      | if (strcmp(mode, 'one value') || strcmp(mode, 'fields of equal size')) && (length(current_widths) > 1),
      |     error('Only one width may be specified for this mode.');
      | elseif strcmp(mode, 'fields of arbitrary size')
      |     current_names = textscan(strtrim(strrep(strrep(get_param(blk, 'names'), ']', ''), '[', '')), '%s');
      |     current_names = current_names{1};
      |     numios = length(current_names);
      |     if length(current_widths) ~= numios,
      |         error('%d field names specified, but %d widths?', numios, length(current_widths));
      |     end
      | end
      | total_width = 0;
      | for ctr = 1 : length(current_widths),
      |     total_width = total_width + current_widths(ctr);
      | end
      | if total_width > 32,
      |     error('Total width must be 32 or less, set to %d.', total_width);
      | end
      mask Callback arith_types:
      | blk = gcb;
      | mode = get_param(blk, 'mode');
      | current_types = eval(get_param(blk, 'arith_types'));
      | numios = length(current_types);
      | if (strcmp(mode, 'one value') || strcmp(mode, 'fields of equal size')) && (length(current_types) > 1),
      |     error('Only one type may be specified for this mode.');
      | elseif strcmp(mode, 'fields of arbitrary size')
      |     current_names = textscan(strtrim(strrep(strrep(get_param(blk, 'names'), ']', ''), '[', '')), '%s');
      |     current_names = current_names{1};
      |     numios = length(current_names);
      |     if length(current_types) ~= numios,
      |         error('%d field names specified, but %d types?', numios, length(current_types));
      |     end
      | end
      | problem = 0;
      | for ctr = 1 : numios,
      |     t = current_types(ctr);
      |     if (t < 0) || (t > 2),
      |         problem = t;
      |         ctr = numios + 1;
      |     end
      | end
      | if problem ~= 0,
      |     error('Type cannot be %i, must be 0, 1 or 2.', problem);
      | end
      mask Callback bin_pts:
      | blk = gcb;
      | mode = get_param(blk, 'mode');
      | current_bins = eval(get_param(blk, 'bin_pts'));
      | if (strcmp(mode, 'one value') || strcmp(mode, 'fields of equal size')) && (length(current_bins) > 1),
      |     error('Only one binary pt may be specified for this mode.');
      | elseif strcmp(mode, 'fields of arbitrary size')
      |     current_names = textscan(strtrim(strrep(strrep(get_param(blk, 'names'), ']', ''), '[', '')), '%s');
      |     current_names = current_names{1};
      |     numios = length(current_names);
      |     if length(current_bins) ~= numios,
      |         error('%d field names specified, but %d binary pts?', numios, length(current_bins));
      |     end
      | end
  vacccnt0 : Subsystem  Tag=xps:sw_reg  AncestorBlock=xps_library/software register  mask(swreg){mode=one value, io_dir=To Processor, io_delay=1, sample_period=1, names=reg, bitwidths=16, arith_types=0, bin_pts=0, sim_port=off, show_format=off}
      mask prompts: io_dir "I/O direction"; io_delay "I/O delay"; sample_period "Sample period"; names "Name:"; bitwidths "Bitwidth:"; arith_types "Type (ufix=0, fix=1, bool=2):"; bin_pts "Binary pt:"; sim_port "Provide sim input/output?"; show_format "Print format string?"
      mask init:
      | swreg_init(gcb)
      settings: AttributesFormatString=1output
      mask TypeOptions mode: one value | fields of equal size | fields of arbitrary size
      mask Callback mode: swreg_cb(gcb);
      mask TypeOptions io_dir: To Processor | From Processor
      mask Callback io_dir:
      | mask_enables = get_param(gcb, 'MaskEnables');
      | mask_names = get_param(gcb, 'MaskNames');
      | if strcmp(get_param(gcb, 'io_dir'), 'To Processor'),
      |     mask_enables{ismember(mask_names, 'sample_period')} = 'off';
      | else
      |     mask_enables{ismember(mask_names, 'sample_period')} = 'on';
      | end
      | set_param(gcb, 'MaskEnables', mask_enables);
      mask Callback bitwidths:
      | blk = gcb;
      | mode = get_param(blk, 'mode');
      | current_widths = eval(get_param(blk, 'bitwidths'));
      | if (strcmp(mode, 'one value') || strcmp(mode, 'fields of equal size')) && (length(current_widths) > 1),
      |     error('Only one width may be specified for this mode.');
      | elseif strcmp(mode, 'fields of arbitrary size')
      |     current_names = textscan(strtrim(strrep(strrep(get_param(blk, 'names'), ']', ''), '[', '')), '%s');
      |     current_names = current_names{1};
      |     numios = length(current_names);
      |     if length(current_widths) ~= numios,
      |         error('%d field names specified, but %d widths?', numios, length(current_widths));
      |     end
      | end
      | total_width = 0;
      | for ctr = 1 : length(current_widths),
      |     total_width = total_width + current_widths(ctr);
      | end
      | if total_width > 32,
      |     error('Total width must be 32 or less, set to %d.', total_width);
      | end
      mask Callback arith_types:
      | blk = gcb;
      | mode = get_param(blk, 'mode');
      | current_types = eval(get_param(blk, 'arith_types'));
      | numios = length(current_types);
      | if (strcmp(mode, 'one value') || strcmp(mode, 'fields of equal size')) && (length(current_types) > 1),
      |     error('Only one type may be specified for this mode.');
      | elseif strcmp(mode, 'fields of arbitrary size')
      |     current_names = textscan(strtrim(strrep(strrep(get_param(blk, 'names'), ']', ''), '[', '')), '%s');
      |     current_names = current_names{1};
      |     numios = length(current_names);
      |     if length(current_types) ~= numios,
      |         error('%d field names specified, but %d types?', numios, length(current_types));
      |     end
      | end
      | problem = 0;
      | for ctr = 1 : numios,
      |     t = current_types(ctr);
      |     if (t < 0) || (t > 2),
      |         problem = t;
      |         ctr = numios + 1;
      |     end
      | end
      | if problem ~= 0,
      |     error('Type cannot be %i, must be 0, 1 or 2.', problem);
      | end
      mask Callback bin_pts:
      | blk = gcb;
      | mode = get_param(blk, 'mode');
      | current_bins = eval(get_param(blk, 'bin_pts'));
      | if (strcmp(mode, 'one value') || strcmp(mode, 'fields of equal size')) && (length(current_bins) > 1),
      |     error('Only one binary pt may be specified for this mode.');
      | elseif strcmp(mode, 'fields of arbitrary size')
      |     current_names = textscan(strtrim(strrep(strrep(get_param(blk, 'names'), ']', ''), '[', '')), '%s');
      |     current_names = current_names{1};
      |     numios = length(current_names);
      |     if length(current_bins) ~= numios,
      |         error('%d field names specified, but %d binary pts?', numios, length(current_bins));
      |     end
      | end
  vacccnt1 : Subsystem  Tag=xps:sw_reg  AncestorBlock=xps_library/software register  mask(swreg){mode=one value, io_dir=To Processor, io_delay=1, sample_period=1, names=reg, bitwidths=16, arith_types=0, bin_pts=0, sim_port=off, show_format=off}
      mask prompts: io_dir "I/O direction"; io_delay "I/O delay"; sample_period "Sample period"; names "Name:"; bitwidths "Bitwidth:"; arith_types "Type (ufix=0, fix=1, bool=2):"; bin_pts "Binary pt:"; sim_port "Provide sim input/output?"; show_format "Print format string?"
      mask init:
      | swreg_init(gcb)
      settings: AttributesFormatString=1output
      mask TypeOptions mode: one value | fields of equal size | fields of arbitrary size
      mask Callback mode: swreg_cb(gcb);
      mask TypeOptions io_dir: To Processor | From Processor
      mask Callback io_dir:
      | mask_enables = get_param(gcb, 'MaskEnables');
      | mask_names = get_param(gcb, 'MaskNames');
      | if strcmp(get_param(gcb, 'io_dir'), 'To Processor'),
      |     mask_enables{ismember(mask_names, 'sample_period')} = 'off';
      | else
      |     mask_enables{ismember(mask_names, 'sample_period')} = 'on';
      | end
      | set_param(gcb, 'MaskEnables', mask_enables);
      mask Callback bitwidths:
      | blk = gcb;
      | mode = get_param(blk, 'mode');
      | current_widths = eval(get_param(blk, 'bitwidths'));
      | if (strcmp(mode, 'one value') || strcmp(mode, 'fields of equal size')) && (length(current_widths) > 1),
      |     error('Only one width may be specified for this mode.');
      | elseif strcmp(mode, 'fields of arbitrary size')
      |     current_names = textscan(strtrim(strrep(strrep(get_param(blk, 'names'), ']', ''), '[', '')), '%s');
      |     current_names = current_names{1};
      |     numios = length(current_names);
      |     if length(current_widths) ~= numios,
      |         error('%d field names specified, but %d widths?', numios, length(current_widths));
      |     end
      | end
      | total_width = 0;
      | for ctr = 1 : length(current_widths),
      |     total_width = total_width + current_widths(ctr);
      | end
      | if total_width > 32,
      |     error('Total width must be 32 or less, set to %d.', total_width);
      | end
      mask Callback arith_types:
      | blk = gcb;
      | mode = get_param(blk, 'mode');
      | current_types = eval(get_param(blk, 'arith_types'));
      | numios = length(current_types);
      | if (strcmp(mode, 'one value') || strcmp(mode, 'fields of equal size')) && (length(current_types) > 1),
      |     error('Only one type may be specified for this mode.');
      | elseif strcmp(mode, 'fields of arbitrary size')
      |     current_names = textscan(strtrim(strrep(strrep(get_param(blk, 'names'), ']', ''), '[', '')), '%s');
      |     current_names = current_names{1};
      |     numios = length(current_names);
      |     if length(current_types) ~= numios,
      |         error('%d field names specified, but %d types?', numios, length(current_types));
      |     end
      | end
      | problem = 0;
      | for ctr = 1 : numios,
      |     t = current_types(ctr);
      |     if (t < 0) || (t > 2),
      |         problem = t;
      |         ctr = numios + 1;
      |     end
      | end
      | if problem ~= 0,
      |     error('Type cannot be %i, must be 0, 1 or 2.', problem);
      | end
      mask Callback bin_pts:
      | blk = gcb;
      | mode = get_param(blk, 'mode');
      | current_bins = eval(get_param(blk, 'bin_pts'));
      | if (strcmp(mode, 'one value') || strcmp(mode, 'fields of equal size')) && (length(current_bins) > 1),
      |     error('Only one binary pt may be specified for this mode.');
      | elseif strcmp(mode, 'fields of arbitrary size')
      |     current_names = textscan(strtrim(strrep(strrep(get_param(blk, 'names'), ']', ''), '[', '')), '%s');
      |     current_names = current_names{1};
      |     numios = length(current_names);
      |     if length(current_bins) ~= numios,
      |         error('%d field names specified, but %d binary pts?', numios, length(current_bins));
      |     end
      | end
  vacccnt2 : Subsystem  Tag=xps:sw_reg  AncestorBlock=xps_library/software register  mask(swreg){mode=one value, io_dir=To Processor, io_delay=1, sample_period=1, names=reg, bitwidths=16, arith_types=0, bin_pts=0, sim_port=off, show_format=off}
      mask prompts: io_dir "I/O direction"; io_delay "I/O delay"; sample_period "Sample period"; names "Name:"; bitwidths "Bitwidth:"; arith_types "Type (ufix=0, fix=1, bool=2):"; bin_pts "Binary pt:"; sim_port "Provide sim input/output?"; show_format "Print format string?"
      mask init:
      | swreg_init(gcb)
      settings: AttributesFormatString=1output
      mask TypeOptions mode: one value | fields of equal size | fields of arbitrary size
      mask Callback mode: swreg_cb(gcb);
      mask TypeOptions io_dir: To Processor | From Processor
      mask Callback io_dir:
      | mask_enables = get_param(gcb, 'MaskEnables');
      | mask_names = get_param(gcb, 'MaskNames');
      | if strcmp(get_param(gcb, 'io_dir'), 'To Processor'),
      |     mask_enables{ismember(mask_names, 'sample_period')} = 'off';
      | else
      |     mask_enables{ismember(mask_names, 'sample_period')} = 'on';
      | end
      | set_param(gcb, 'MaskEnables', mask_enables);
      mask Callback bitwidths:
      | blk = gcb;
      | mode = get_param(blk, 'mode');
      | current_widths = eval(get_param(blk, 'bitwidths'));
      | if (strcmp(mode, 'one value') || strcmp(mode, 'fields of equal size')) && (length(current_widths) > 1),
      |     error('Only one width may be specified for this mode.');
      | elseif strcmp(mode, 'fields of arbitrary size')
      |     current_names = textscan(strtrim(strrep(strrep(get_param(blk, 'names'), ']', ''), '[', '')), '%s');
      |     current_names = current_names{1};
      |     numios = length(current_names);
      |     if length(current_widths) ~= numios,
      |         error('%d field names specified, but %d widths?', numios, length(current_widths));
      |     end
      | end
      | total_width = 0;
      | for ctr = 1 : length(current_widths),
      |     total_width = total_width + current_widths(ctr);
      | end
      | if total_width > 32,
      |     error('Total width must be 32 or less, set to %d.', total_width);
      | end
      mask Callback arith_types:
      | blk = gcb;
      | mode = get_param(blk, 'mode');
      | current_types = eval(get_param(blk, 'arith_types'));
      | numios = length(current_types);
      | if (strcmp(mode, 'one value') || strcmp(mode, 'fields of equal size')) && (length(current_types) > 1),
      |     error('Only one type may be specified for this mode.');
      | elseif strcmp(mode, 'fields of arbitrary size')
      |     current_names = textscan(strtrim(strrep(strrep(get_param(blk, 'names'), ']', ''), '[', '')), '%s');
      |     current_names = current_names{1};
      |     numios = length(current_names);
      |     if length(current_types) ~= numios,
      |         error('%d field names specified, but %d types?', numios, length(current_types));
      |     end
      | end
      | problem = 0;
      | for ctr = 1 : numios,
      |     t = current_types(ctr);
      |     if (t < 0) || (t > 2),
      |         problem = t;
      |         ctr = numios + 1;
      |     end
      | end
      | if problem ~= 0,
      |     error('Type cannot be %i, must be 0, 1 or 2.', problem);
      | end
      mask Callback bin_pts:
      | blk = gcb;
      | mode = get_param(blk, 'mode');
      | current_bins = eval(get_param(blk, 'bin_pts'));
      | if (strcmp(mode, 'one value') || strcmp(mode, 'fields of equal size')) && (length(current_bins) > 1),
      |     error('Only one binary pt may be specified for this mode.');
      | elseif strcmp(mode, 'fields of arbitrary size')
      |     current_names = textscan(strtrim(strrep(strrep(get_param(blk, 'names'), ']', ''), '[', '')), '%s');
      |     current_names = current_names{1};
      |     numios = length(current_names);
      |     if length(current_bins) ~= numios,
      |         error('%d field names specified, but %d binary pts?', numios, length(current_bins));
      |     end
      | end
  vacccnt3 : Subsystem  Tag=xps:sw_reg  AncestorBlock=xps_library/software register  mask(swreg){mode=one value, io_dir=To Processor, io_delay=1, sample_period=1, names=reg, bitwidths=16, arith_types=0, bin_pts=0, sim_port=off, show_format=off}
      mask prompts: io_dir "I/O direction"; io_delay "I/O delay"; sample_period "Sample period"; names "Name:"; bitwidths "Bitwidth:"; arith_types "Type (ufix=0, fix=1, bool=2):"; bin_pts "Binary pt:"; sim_port "Provide sim input/output?"; show_format "Print format string?"
      mask init:
      | swreg_init(gcb)
      settings: AttributesFormatString=1output
      mask TypeOptions mode: one value | fields of equal size | fields of arbitrary size
      mask Callback mode: swreg_cb(gcb);
      mask TypeOptions io_dir: To Processor | From Processor
      mask Callback io_dir:
      | mask_enables = get_param(gcb, 'MaskEnables');
      | mask_names = get_param(gcb, 'MaskNames');
      | if strcmp(get_param(gcb, 'io_dir'), 'To Processor'),
      |     mask_enables{ismember(mask_names, 'sample_period')} = 'off';
      | else
      |     mask_enables{ismember(mask_names, 'sample_period')} = 'on';
      | end
      | set_param(gcb, 'MaskEnables', mask_enables);
      mask Callback bitwidths:
      | blk = gcb;
      | mode = get_param(blk, 'mode');
      | current_widths = eval(get_param(blk, 'bitwidths'));
      | if (strcmp(mode, 'one value') || strcmp(mode, 'fields of equal size')) && (length(current_widths) > 1),
      |     error('Only one width may be specified for this mode.');
      | elseif strcmp(mode, 'fields of arbitrary size')
      |     current_names = textscan(strtrim(strrep(strrep(get_param(blk, 'names'), ']', ''), '[', '')), '%s');
      |     current_names = current_names{1};
      |     numios = length(current_names);
      |     if length(current_widths) ~= numios,
      |         error('%d field names specified, but %d widths?', numios, length(current_widths));
      |     end
      | end
      | total_width = 0;
      | for ctr = 1 : length(current_widths),
      |     total_width = total_width + current_widths(ctr);
      | end
      | if total_width > 32,
      |     error('Total width must be 32 or less, set to %d.', total_width);
      | end
      mask Callback arith_types:
      | blk = gcb;
      | mode = get_param(blk, 'mode');
      | current_types = eval(get_param(blk, 'arith_types'));
      | numios = length(current_types);
      | if (strcmp(mode, 'one value') || strcmp(mode, 'fields of equal size')) && (length(current_types) > 1),
      |     error('Only one type may be specified for this mode.');
      | elseif strcmp(mode, 'fields of arbitrary size')
      |     current_names = textscan(strtrim(strrep(strrep(get_param(blk, 'names'), ']', ''), '[', '')), '%s');
      |     current_names = current_names{1};
      |     numios = length(current_names);
      |     if length(current_types) ~= numios,
      |         error('%d field names specified, but %d types?', numios, length(current_types));
      |     end
      | end
      | problem = 0;
      | for ctr = 1 : numios,
      |     t = current_types(ctr);
      |     if (t < 0) || (t > 2),
      |         problem = t;
      |         ctr = numios + 1;
      |     end
      | end
      | if problem ~= 0,
      |     error('Type cannot be %i, must be 0, 1 or 2.', problem);
      | end
      mask Callback bin_pts:
      | blk = gcb;
      | mode = get_param(blk, 'mode');
      | current_bins = eval(get_param(blk, 'bin_pts'));
      | if (strcmp(mode, 'one value') || strcmp(mode, 'fields of equal size')) && (length(current_bins) > 1),
      |     error('Only one binary pt may be specified for this mode.');
      | elseif strcmp(mode, 'fields of arbitrary size')
      |     current_names = textscan(strtrim(strrep(strrep(get_param(blk, 'names'), ']', ''), '[', '')), '%s');
      |     current_names = current_names{1};
      |     numios = length(current_names);
      |     if length(current_bins) ~= numios,
      |         error('%d field names specified, but %d binary pts?', numios, length(current_bins));
      |     end
      | end
  vaccerr0 : Subsystem  Tag=xps:sw_reg  AncestorBlock=xps_library/software register  mask(swreg){mode=one value, io_dir=To Processor, io_delay=1, sample_period=1, names=reg, bitwidths=16, arith_types=0, bin_pts=0, sim_port=off, show_format=off}
      mask prompts: io_dir "I/O direction"; io_delay "I/O delay"; sample_period "Sample period"; names "Name:"; bitwidths "Bitwidth:"; arith_types "Type (ufix=0, fix=1, bool=2):"; bin_pts "Binary pt:"; sim_port "Provide sim input/output?"; show_format "Print format string?"
      mask init:
      | swreg_init(gcb)
      settings: AttributesFormatString=1output
      mask TypeOptions mode: one value | fields of equal size | fields of arbitrary size
      mask Callback mode: swreg_cb(gcb);
      mask TypeOptions io_dir: To Processor | From Processor
      mask Callback io_dir:
      | mask_enables = get_param(gcb, 'MaskEnables');
      | mask_names = get_param(gcb, 'MaskNames');
      | if strcmp(get_param(gcb, 'io_dir'), 'To Processor'),
      |     mask_enables{ismember(mask_names, 'sample_period')} = 'off';
      | else
      |     mask_enables{ismember(mask_names, 'sample_period')} = 'on';
      | end
      | set_param(gcb, 'MaskEnables', mask_enables);
      mask Callback bitwidths:
      | blk = gcb;
      | mode = get_param(blk, 'mode');
      | current_widths = eval(get_param(blk, 'bitwidths'));
      | if (strcmp(mode, 'one value') || strcmp(mode, 'fields of equal size')) && (length(current_widths) > 1),
      |     error('Only one width may be specified for this mode.');
      | elseif strcmp(mode, 'fields of arbitrary size')
      |     current_names = textscan(strtrim(strrep(strrep(get_param(blk, 'names'), ']', ''), '[', '')), '%s');
      |     current_names = current_names{1};
      |     numios = length(current_names);
      |     if length(current_widths) ~= numios,
      |         error('%d field names specified, but %d widths?', numios, length(current_widths));
      |     end
      | end
      | total_width = 0;
      | for ctr = 1 : length(current_widths),
      |     total_width = total_width + current_widths(ctr);
      | end
      | if total_width > 32,
      |     error('Total width must be 32 or less, set to %d.', total_width);
      | end
      mask Callback arith_types:
      | blk = gcb;
      | mode = get_param(blk, 'mode');
      | current_types = eval(get_param(blk, 'arith_types'));
      | numios = length(current_types);
      | if (strcmp(mode, 'one value') || strcmp(mode, 'fields of equal size')) && (length(current_types) > 1),
      |     error('Only one type may be specified for this mode.');
      | elseif strcmp(mode, 'fields of arbitrary size')
      |     current_names = textscan(strtrim(strrep(strrep(get_param(blk, 'names'), ']', ''), '[', '')), '%s');
      |     current_names = current_names{1};
      |     numios = length(current_names);
      |     if length(current_types) ~= numios,
      |         error('%d field names specified, but %d types?', numios, length(current_types));
      |     end
      | end
      | problem = 0;
      | for ctr = 1 : numios,
      |     t = current_types(ctr);
      |     if (t < 0) || (t > 2),
      |         problem = t;
      |         ctr = numios + 1;
      |     end
      | end
      | if problem ~= 0,
      |     error('Type cannot be %i, must be 0, 1 or 2.', problem);
      | end
      mask Callback bin_pts:
      | blk = gcb;
      | mode = get_param(blk, 'mode');
      | current_bins = eval(get_param(blk, 'bin_pts'));
      | if (strcmp(mode, 'one value') || strcmp(mode, 'fields of equal size')) && (length(current_bins) > 1),
      |     error('Only one binary pt may be specified for this mode.');
      | elseif strcmp(mode, 'fields of arbitrary size')
      |     current_names = textscan(strtrim(strrep(strrep(get_param(blk, 'names'), ']', ''), '[', '')), '%s');
      |     current_names = current_names{1};
      |     numios = length(current_names);
      |     if length(current_bins) ~= numios,
      |         error('%d field names specified, but %d binary pts?', numios, length(current_bins));
      |     end
      | end
  vaccerr1 : Subsystem  Tag=xps:sw_reg  AncestorBlock=xps_library/software register  mask(swreg){mode=one value, io_dir=To Processor, io_delay=1, sample_period=1, names=reg, bitwidths=16, arith_types=0, bin_pts=0, sim_port=off, show_format=off}
      mask prompts: io_dir "I/O direction"; io_delay "I/O delay"; sample_period "Sample period"; names "Name:"; bitwidths "Bitwidth:"; arith_types "Type (ufix=0, fix=1, bool=2):"; bin_pts "Binary pt:"; sim_port "Provide sim input/output?"; show_format "Print format string?"
      mask init:
      | swreg_init(gcb)
      settings: AttributesFormatString=1output
      mask TypeOptions mode: one value | fields of equal size | fields of arbitrary size
      mask Callback mode: swreg_cb(gcb);
      mask TypeOptions io_dir: To Processor | From Processor
      mask Callback io_dir:
      | mask_enables = get_param(gcb, 'MaskEnables');
      | mask_names = get_param(gcb, 'MaskNames');
      | if strcmp(get_param(gcb, 'io_dir'), 'To Processor'),
      |     mask_enables{ismember(mask_names, 'sample_period')} = 'off';
      | else
      |     mask_enables{ismember(mask_names, 'sample_period')} = 'on';
      | end
      | set_param(gcb, 'MaskEnables', mask_enables);
      mask Callback bitwidths:
      | blk = gcb;
      | mode = get_param(blk, 'mode');
      | current_widths = eval(get_param(blk, 'bitwidths'));
      | if (strcmp(mode, 'one value') || strcmp(mode, 'fields of equal size')) && (length(current_widths) > 1),
      |     error('Only one width may be specified for this mode.');
      | elseif strcmp(mode, 'fields of arbitrary size')
      |     current_names = textscan(strtrim(strrep(strrep(get_param(blk, 'names'), ']', ''), '[', '')), '%s');
      |     current_names = current_names{1};
      |     numios = length(current_names);
      |     if length(current_widths) ~= numios,
      |         error('%d field names specified, but %d widths?', numios, length(current_widths));
      |     end
      | end
      | total_width = 0;
      | for ctr = 1 : length(current_widths),
      |     total_width = total_width + current_widths(ctr);
      | end
      | if total_width > 32,
      |     error('Total width must be 32 or less, set to %d.', total_width);
      | end
      mask Callback arith_types:
      | blk = gcb;
      | mode = get_param(blk, 'mode');
      | current_types = eval(get_param(blk, 'arith_types'));
      | numios = length(current_types);
      | if (strcmp(mode, 'one value') || strcmp(mode, 'fields of equal size')) && (length(current_types) > 1),
      |     error('Only one type may be specified for this mode.');
      | elseif strcmp(mode, 'fields of arbitrary size')
      |     current_names = textscan(strtrim(strrep(strrep(get_param(blk, 'names'), ']', ''), '[', '')), '%s');
      |     current_names = current_names{1};
      |     numios = length(current_names);
      |     if length(current_types) ~= numios,
      |         error('%d field names specified, but %d types?', numios, length(current_types));
      |     end
      | end
      | problem = 0;
      | for ctr = 1 : numios,
      |     t = current_types(ctr);
      |     if (t < 0) || (t > 2),
      |         problem = t;
      |         ctr = numios + 1;
      |     end
      | end
      | if problem ~= 0,
      |     error('Type cannot be %i, must be 0, 1 or 2.', problem);
      | end
      mask Callback bin_pts:
      | blk = gcb;
      | mode = get_param(blk, 'mode');
      | current_bins = eval(get_param(blk, 'bin_pts'));
      | if (strcmp(mode, 'one value') || strcmp(mode, 'fields of equal size')) && (length(current_bins) > 1),
      |     error('Only one binary pt may be specified for this mode.');
      | elseif strcmp(mode, 'fields of arbitrary size')
      |     current_names = textscan(strtrim(strrep(strrep(get_param(blk, 'names'), ']', ''), '[', '')), '%s');
      |     current_names = current_names{1};
      |     numios = length(current_names);
      |     if length(current_bins) ~= numios,
      |         error('%d field names specified, but %d binary pts?', numios, length(current_bins));
      |     end
      | end
  vaccerr2 : Subsystem  Tag=xps:sw_reg  AncestorBlock=xps_library/software register  mask(swreg){mode=one value, io_dir=To Processor, io_delay=1, sample_period=1, names=reg, bitwidths=16, arith_types=0, bin_pts=0, sim_port=off, show_format=off}
      mask prompts: io_dir "I/O direction"; io_delay "I/O delay"; sample_period "Sample period"; names "Name:"; bitwidths "Bitwidth:"; arith_types "Type (ufix=0, fix=1, bool=2):"; bin_pts "Binary pt:"; sim_port "Provide sim input/output?"; show_format "Print format string?"
      mask init:
      | swreg_init(gcb)
      settings: AttributesFormatString=1output
      mask TypeOptions mode: one value | fields of equal size | fields of arbitrary size
      mask Callback mode: swreg_cb(gcb);
      mask TypeOptions io_dir: To Processor | From Processor
      mask Callback io_dir:
      | mask_enables = get_param(gcb, 'MaskEnables');
      | mask_names = get_param(gcb, 'MaskNames');
      | if strcmp(get_param(gcb, 'io_dir'), 'To Processor'),
      |     mask_enables{ismember(mask_names, 'sample_period')} = 'off';
      | else
      |     mask_enables{ismember(mask_names, 'sample_period')} = 'on';
      | end
      | set_param(gcb, 'MaskEnables', mask_enables);
      mask Callback bitwidths:
      | blk = gcb;
      | mode = get_param(blk, 'mode');
      | current_widths = eval(get_param(blk, 'bitwidths'));
      | if (strcmp(mode, 'one value') || strcmp(mode, 'fields of equal size')) && (length(current_widths) > 1),
      |     error('Only one width may be specified for this mode.');
      | elseif strcmp(mode, 'fields of arbitrary size')
      |     current_names = textscan(strtrim(strrep(strrep(get_param(blk, 'names'), ']', ''), '[', '')), '%s');
      |     current_names = current_names{1};
      |     numios = length(current_names);
      |     if length(current_widths) ~= numios,
      |         error('%d field names specified, but %d widths?', numios, length(current_widths));
      |     end
      | end
      | total_width = 0;
      | for ctr = 1 : length(current_widths),
      |     total_width = total_width + current_widths(ctr);
      | end
      | if total_width > 32,
      |     error('Total width must be 32 or less, set to %d.', total_width);
      | end
      mask Callback arith_types:
      | blk = gcb;
      | mode = get_param(blk, 'mode');
      | current_types = eval(get_param(blk, 'arith_types'));
      | numios = length(current_types);
      | if (strcmp(mode, 'one value') || strcmp(mode, 'fields of equal size')) && (length(current_types) > 1),
      |     error('Only one type may be specified for this mode.');
      | elseif strcmp(mode, 'fields of arbitrary size')
      |     current_names = textscan(strtrim(strrep(strrep(get_param(blk, 'names'), ']', ''), '[', '')), '%s');
      |     current_names = current_names{1};
      |     numios = length(current_names);
      |     if length(current_types) ~= numios,
      |         error('%d field names specified, but %d types?', numios, length(current_types));
      |     end
      | end
      | problem = 0;
      | for ctr = 1 : numios,
      |     t = current_types(ctr);
      |     if (t < 0) || (t > 2),
      |         problem = t;
      |         ctr = numios + 1;
      |     end
      | end
      | if problem ~= 0,
      |     error('Type cannot be %i, must be 0, 1 or 2.', problem);
      | end
      mask Callback bin_pts:
      | blk = gcb;
      | mode = get_param(blk, 'mode');
      | current_bins = eval(get_param(blk, 'bin_pts'));
      | if (strcmp(mode, 'one value') || strcmp(mode, 'fields of equal size')) && (length(current_bins) > 1),
      |     error('Only one binary pt may be specified for this mode.');
      | elseif strcmp(mode, 'fields of arbitrary size')
      |     current_names = textscan(strtrim(strrep(strrep(get_param(blk, 'names'), ']', ''), '[', '')), '%s');
      |     current_names = current_names{1};
      |     numios = length(current_names);
      |     if length(current_bins) ~= numios,
      |         error('%d field names specified, but %d binary pts?', numios, length(current_bins));
      |     end
      | end
  vaccerr3 : Subsystem  Tag=xps:sw_reg  AncestorBlock=xps_library/software register  mask(swreg){mode=one value, io_dir=To Processor, io_delay=1, sample_period=1, names=reg, bitwidths=16, arith_types=0, bin_pts=0, sim_port=off, show_format=off}
      mask prompts: io_dir "I/O direction"; io_delay "I/O delay"; sample_period "Sample period"; names "Name:"; bitwidths "Bitwidth:"; arith_types "Type (ufix=0, fix=1, bool=2):"; bin_pts "Binary pt:"; sim_port "Provide sim input/output?"; show_format "Print format string?"
      mask init:
      | swreg_init(gcb)
      settings: AttributesFormatString=1output
      mask TypeOptions mode: one value | fields of equal size | fields of arbitrary size
      mask Callback mode: swreg_cb(gcb);
      mask TypeOptions io_dir: To Processor | From Processor
      mask Callback io_dir:
      | mask_enables = get_param(gcb, 'MaskEnables');
      | mask_names = get_param(gcb, 'MaskNames');
      | if strcmp(get_param(gcb, 'io_dir'), 'To Processor'),
      |     mask_enables{ismember(mask_names, 'sample_period')} = 'off';
      | else
      |     mask_enables{ismember(mask_names, 'sample_period')} = 'on';
      | end
      | set_param(gcb, 'MaskEnables', mask_enables);
      mask Callback bitwidths:
      | blk = gcb;
      | mode = get_param(blk, 'mode');
      | current_widths = eval(get_param(blk, 'bitwidths'));
      | if (strcmp(mode, 'one value') || strcmp(mode, 'fields of equal size')) && (length(current_widths) > 1),
      |     error('Only one width may be specified for this mode.');
      | elseif strcmp(mode, 'fields of arbitrary size')
      |     current_names = textscan(strtrim(strrep(strrep(get_param(blk, 'names'), ']', ''), '[', '')), '%s');
      |     current_names = current_names{1};
      |     numios = length(current_names);
      |     if length(current_widths) ~= numios,
      |         error('%d field names specified, but %d widths?', numios, length(current_widths));
      |     end
      | end
      | total_width = 0;
      | for ctr = 1 : length(current_widths),
      |     total_width = total_width + current_widths(ctr);
      | end
      | if total_width > 32,
      |     error('Total width must be 32 or less, set to %d.', total_width);
      | end
      mask Callback arith_types:
      | blk = gcb;
      | mode = get_param(blk, 'mode');
      | current_types = eval(get_param(blk, 'arith_types'));
      | numios = length(current_types);
      | if (strcmp(mode, 'one value') || strcmp(mode, 'fields of equal size')) && (length(current_types) > 1),
      |     error('Only one type may be specified for this mode.');
      | elseif strcmp(mode, 'fields of arbitrary size')
      |     current_names = textscan(strtrim(strrep(strrep(get_param(blk, 'names'), ']', ''), '[', '')), '%s');
      |     current_names = current_names{1};
      |     numios = length(current_names);
      |     if length(current_types) ~= numios,
      |         error('%d field names specified, but %d types?', numios, length(current_types));
      |     end
      | end
      | problem = 0;
      | for ctr = 1 : numios,
      |     t = current_types(ctr);
      |     if (t < 0) || (t > 2),
      |         problem = t;
      |         ctr = numios + 1;
      |     end
      | end
      | if problem ~= 0,
      |     error('Type cannot be %i, must be 0, 1 or 2.', problem);
      | end
      mask Callback bin_pts:
      | blk = gcb;
      | mode = get_param(blk, 'mode');
      | current_bins = eval(get_param(blk, 'bin_pts'));
      | if (strcmp(mode, 'one value') || strcmp(mode, 'fields of equal size')) && (length(current_bins) > 1),
      |     error('Only one binary pt may be specified for this mode.');
      | elseif strcmp(mode, 'fields of arbitrary size')
      |     current_names = textscan(strtrim(strrep(strrep(get_param(blk, 'names'), ']', ''), '[', '')), '%s');
      |     current_names = current_names{1};
      |     numios = length(current_names);
      |     if length(current_bins) ~= numios,
      |         error('%d field names specified, but %d binary pts?', numios, length(current_bins));
      |     end
      | end
  vaccin_newtvg : Subsystem  Tag=xps:sw_reg  AncestorBlock=xps_library/software register  mask(swreg){mode=one value, io_dir=From Processor, io_delay=0, sample_period=1, names=reg, bitwidths=32, arith_types=0, bin_pts=0, sim_port=off, show_format=on}
      mask prompts: io_dir "I/O direction"; io_delay "I/O delay"; sample_period "Sample period"; names "Name:"; bitwidths "Bitwidth:"; arith_types "Type (ufix=0, fix=1, bool=2):"; bin_pts "Binary pt:"; sim_port "Provide sim input/output?"; show_format "Print format string?"
      mask init:
      | swreg_init(gcb)
      settings: AttributesFormatString=1input:uf32.0,
      mask TypeOptions mode: one value | fields of equal size | fields of arbitrary size
      mask Callback mode: swreg_cb(gcb);
      mask TypeOptions io_dir: To Processor | From Processor
      mask Callback io_dir:
      | mask_enables = get_param(gcb, 'MaskEnables');
      | mask_names = get_param(gcb, 'MaskNames');
      | if strcmp(get_param(gcb, 'io_dir'), 'To Processor'),
      |     mask_enables{ismember(mask_names, 'sample_period')} = 'off';
      | else
      |     mask_enables{ismember(mask_names, 'sample_period')} = 'on';
      | end
      | set_param(gcb, 'MaskEnables', mask_enables);
      mask Callback bitwidths:
      | blk = gcb;
      | mode = get_param(blk, 'mode');
      | current_widths = eval(get_param(blk, 'bitwidths'));
      | if (strcmp(mode, 'one value') || strcmp(mode, 'fields of equal size')) && (length(current_widths) > 1),
      |     error('Only one width may be specified for this mode.');
      | elseif strcmp(mode, 'fields of arbitrary size')
      |     current_names = textscan(strtrim(strrep(strrep(get_param(blk, 'names'), ']', ''), '[', '')), '%s');
      |     current_names = current_names{1};
      |     numios = length(current_names);
      |     if length(current_widths) ~= numios,
      |         error('%d field names specified, but %d widths?', numios, length(current_widths));
      |     end
      | end
      | total_width = 0;
      | for ctr = 1 : length(current_widths),
      |     total_width = total_width + current_widths(ctr);
      | end
      | if total_width > 32,
      |     error('Total width must be 32 or less, set to %d.', total_width);
      | end
      mask Callback arith_types:
      | blk = gcb;
      | mode = get_param(blk, 'mode');
      | current_types = eval(get_param(blk, 'arith_types'));
      | numios = length(current_types);
      | if (strcmp(mode, 'one value') || strcmp(mode, 'fields of equal size')) && (length(current_types) > 1),
      |     error('Only one type may be specified for this mode.');
      | elseif strcmp(mode, 'fields of arbitrary size')
      |     current_names = textscan(strtrim(strrep(strrep(get_param(blk, 'names'), ']', ''), '[', '')), '%s');
      |     current_names = current_names{1};
      |     numios = length(current_names);
      |     if length(current_types) ~= numios,
      |         error('%d field names specified, but %d types?', numios, length(current_types));
      |     end
      | end
      | problem = 0;
      | for ctr = 1 : numios,
      |     t = current_types(ctr);
      |     if (t < 0) || (t > 2),
      |         problem = t;
      |         ctr = numios + 1;
      |     end
      | end
      | if problem ~= 0,
      |     error('Type cannot be %i, must be 0, 1 or 2.', problem);
      | end
      mask Callback bin_pts:
      | blk = gcb;
      | mode = get_param(blk, 'mode');
      | current_bins = eval(get_param(blk, 'bin_pts'));
      | if (strcmp(mode, 'one value') || strcmp(mode, 'fields of equal size')) && (length(current_bins) > 1),
      |     error('Only one binary pt may be specified for this mode.');
      | elseif strcmp(mode, 'fields of arbitrary size')
      |     current_names = textscan(strtrim(strrep(strrep(get_param(blk, 'names'), ']', ''), '[', '')), '%s');
      |     current_names = current_names{1};
      |     numios = length(current_names);
      |     if length(current_bins) ~= numios,
      |         error('%d field names specified, but %d binary pts?', numios, length(current_bins));
      |     end
      | end
  vaccout0 : Subsystem  Tag=xps:sw_reg  AncestorBlock=xps_library/software register  mask(swreg){mode=fields of arbitrary size, io_dir=To Processor, io_delay=1, sample_period=1, names=[ready_cnt eof_cnt], bitwidths=[16 16], arith_types=[0 0], bin_pts=0, sim_port=off, show_format=off}
      mask prompts: io_dir "I/O direction"; io_delay "I/O delay"; sample_period "Sample period"; names "Names [msb ... lsb]:"; bitwidths "Bitwidths [msb ... lsb]:"; arith_types "Types (ufix=0, fix=1, bool=2) [msb ... lsb]:"; bin_pts "Binary pts [msb ... lsb]:"; sim_port "Provide sim input/output?"; show_format "Print format string?"
      mask init:
      | swreg_init(gcb)
      settings: AttributesFormatString=2 outputs
      mask TypeOptions mode: one value | fields of equal size | fields of arbitrary size
      mask Callback mode: swreg_cb(gcb);
      mask TypeOptions io_dir: To Processor | From Processor
      mask Callback io_dir:
      | mask_enables = get_param(gcb, 'MaskEnables');
      | mask_names = get_param(gcb, 'MaskNames');
      | if strcmp(get_param(gcb, 'io_dir'), 'To Processor'),
      |     mask_enables{ismember(mask_names, 'sample_period')} = 'off';
      | else
      |     mask_enables{ismember(mask_names, 'sample_period')} = 'on';
      | end
      | set_param(gcb, 'MaskEnables', mask_enables);
      mask Callback bitwidths:
      | blk = gcb;
      | mode = get_param(blk, 'mode');
      | current_widths = eval(get_param(blk, 'bitwidths'));
      | if (strcmp(mode, 'one value') || strcmp(mode, 'fields of equal size')) && (length(current_widths) > 1),
      |     error('Only one width may be specified for this mode.');
      | elseif strcmp(mode, 'fields of arbitrary size')
      |     current_names = textscan(strtrim(strrep(strrep(get_param(blk, 'names'), ']', ''), '[', '')), '%s');
      |     current_names = current_names{1};
      |     numios = length(current_names);
      |     if length(current_widths) ~= numios,
      |         error('%d field names specified, but %d widths?', numios, length(current_widths));
      |     end
      | end
      | total_width = 0;
      | for ctr = 1 : length(current_widths),
      |     total_width = total_width + current_widths(ctr);
      | end
      | if total_width > 32,
      |     error('Total width must be 32 or less, set to %d.', total_width);
      | end
      mask Callback arith_types:
      | blk = gcb;
      | mode = get_param(blk, 'mode');
      | current_types = eval(get_param(blk, 'arith_types'));
      | numios = length(current_types);
      | if (strcmp(mode, 'one value') || strcmp(mode, 'fields of equal size')) && (length(current_types) > 1),
      |     error('Only one type may be specified for this mode.');
      | elseif strcmp(mode, 'fields of arbitrary size')
      |     current_names = textscan(strtrim(strrep(strrep(get_param(blk, 'names'), ']', ''), '[', '')), '%s');
      |     current_names = current_names{1};
      |     numios = length(current_names);
      |     if length(current_types) ~= numios,
      |         error('%d field names specified, but %d types?', numios, length(current_types));
      |     end
      | end
      | problem = 0;
      | for ctr = 1 : numios,
      |     t = current_types(ctr);
      |     if (t < 0) || (t > 2),
      |         problem = t;
      |         ctr = numios + 1;
      |     end
      | end
      | if problem ~= 0,
      |     error('Type cannot be %i, must be 0, 1 or 2.', problem);
      | end
      mask Callback bin_pts:
      | blk = gcb;
      | mode = get_param(blk, 'mode');
      | current_bins = eval(get_param(blk, 'bin_pts'));
      | if (strcmp(mode, 'one value') || strcmp(mode, 'fields of equal size')) && (length(current_bins) > 1),
      |     error('Only one binary pt may be specified for this mode.');
      | elseif strcmp(mode, 'fields of arbitrary size')
      |     current_names = textscan(strtrim(strrep(strrep(get_param(blk, 'names'), ']', ''), '[', '')), '%s');
      |     current_names = current_names{1};
      |     numios = length(current_names);
      |     if length(current_bins) ~= numios,
      |         error('%d field names specified, but %d binary pts?', numios, length(current_bins));
      |     end
      | end
  vaccout1 : Subsystem  Tag=xps:sw_reg  AncestorBlock=xps_library/software register  mask(swreg){mode=fields of arbitrary size, io_dir=To Processor, io_delay=1, sample_period=1, names=[ready_cnt eof_cnt], bitwidths=[16 16], arith_types=[0 0], bin_pts=0, sim_port=off, show_format=off}
      mask prompts: io_dir "I/O direction"; io_delay "I/O delay"; sample_period "Sample period"; names "Names [msb ... lsb]:"; bitwidths "Bitwidths [msb ... lsb]:"; arith_types "Types (ufix=0, fix=1, bool=2) [msb ... lsb]:"; bin_pts "Binary pts [msb ... lsb]:"; sim_port "Provide sim input/output?"; show_format "Print format string?"
      mask init:
      | swreg_init(gcb)
      settings: AttributesFormatString=2 outputs
      mask TypeOptions mode: one value | fields of equal size | fields of arbitrary size
      mask Callback mode: swreg_cb(gcb);
      mask TypeOptions io_dir: To Processor | From Processor
      mask Callback io_dir:
      | mask_enables = get_param(gcb, 'MaskEnables');
      | mask_names = get_param(gcb, 'MaskNames');
      | if strcmp(get_param(gcb, 'io_dir'), 'To Processor'),
      |     mask_enables{ismember(mask_names, 'sample_period')} = 'off';
      | else
      |     mask_enables{ismember(mask_names, 'sample_period')} = 'on';
      | end
      | set_param(gcb, 'MaskEnables', mask_enables);
      mask Callback bitwidths:
      | blk = gcb;
      | mode = get_param(blk, 'mode');
      | current_widths = eval(get_param(blk, 'bitwidths'));
      | if (strcmp(mode, 'one value') || strcmp(mode, 'fields of equal size')) && (length(current_widths) > 1),
      |     error('Only one width may be specified for this mode.');
      | elseif strcmp(mode, 'fields of arbitrary size')
      |     current_names = textscan(strtrim(strrep(strrep(get_param(blk, 'names'), ']', ''), '[', '')), '%s');
      |     current_names = current_names{1};
      |     numios = length(current_names);
      |     if length(current_widths) ~= numios,
      |         error('%d field names specified, but %d widths?', numios, length(current_widths));
      |     end
      | end
      | total_width = 0;
      | for ctr = 1 : length(current_widths),
      |     total_width = total_width + current_widths(ctr);
      | end
      | if total_width > 32,
      |     error('Total width must be 32 or less, set to %d.', total_width);
      | end
      mask Callback arith_types:
      | blk = gcb;
      | mode = get_param(blk, 'mode');
      | current_types = eval(get_param(blk, 'arith_types'));
      | numios = length(current_types);
      | if (strcmp(mode, 'one value') || strcmp(mode, 'fields of equal size')) && (length(current_types) > 1),
      |     error('Only one type may be specified for this mode.');
      | elseif strcmp(mode, 'fields of arbitrary size')
      |     current_names = textscan(strtrim(strrep(strrep(get_param(blk, 'names'), ']', ''), '[', '')), '%s');
      |     current_names = current_names{1};
      |     numios = length(current_names);
      |     if length(current_types) ~= numios,
      |         error('%d field names specified, but %d types?', numios, length(current_types));
      |     end
      | end
      | problem = 0;
      | for ctr = 1 : numios,
      |     t = current_types(ctr);
      |     if (t < 0) || (t > 2),
      |         problem = t;
      |         ctr = numios + 1;
      |     end
      | end
      | if problem ~= 0,
      |     error('Type cannot be %i, must be 0, 1 or 2.', problem);
      | end
      mask Callback bin_pts:
      | blk = gcb;
      | mode = get_param(blk, 'mode');
      | current_bins = eval(get_param(blk, 'bin_pts'));
      | if (strcmp(mode, 'one value') || strcmp(mode, 'fields of equal size')) && (length(current_bins) > 1),
      |     error('Only one binary pt may be specified for this mode.');
      | elseif strcmp(mode, 'fields of arbitrary size')
      |     current_names = textscan(strtrim(strrep(strrep(get_param(blk, 'names'), ']', ''), '[', '')), '%s');
      |     current_names = current_names{1};
      |     numios = length(current_names);
      |     if length(current_bins) ~= numios,
      |         error('%d field names specified, but %d binary pts?', numios, length(current_bins));
      |     end
      | end
  vaccout2 : Subsystem  Tag=xps:sw_reg  AncestorBlock=xps_library/software register  mask(swreg){mode=fields of arbitrary size, io_dir=To Processor, io_delay=1, sample_period=1, names=[ready_cnt eof_cnt], bitwidths=[16 16], arith_types=[0 0], bin_pts=0, sim_port=off, show_format=off}
      mask prompts: io_dir "I/O direction"; io_delay "I/O delay"; sample_period "Sample period"; names "Names [msb ... lsb]:"; bitwidths "Bitwidths [msb ... lsb]:"; arith_types "Types (ufix=0, fix=1, bool=2) [msb ... lsb]:"; bin_pts "Binary pts [msb ... lsb]:"; sim_port "Provide sim input/output?"; show_format "Print format string?"
      mask init:
      | swreg_init(gcb)
      settings: AttributesFormatString=2 outputs
      mask TypeOptions mode: one value | fields of equal size | fields of arbitrary size
      mask Callback mode: swreg_cb(gcb);
      mask TypeOptions io_dir: To Processor | From Processor
      mask Callback io_dir:
      | mask_enables = get_param(gcb, 'MaskEnables');
      | mask_names = get_param(gcb, 'MaskNames');
      | if strcmp(get_param(gcb, 'io_dir'), 'To Processor'),
      |     mask_enables{ismember(mask_names, 'sample_period')} = 'off';
      | else
      |     mask_enables{ismember(mask_names, 'sample_period')} = 'on';
      | end
      | set_param(gcb, 'MaskEnables', mask_enables);
      mask Callback bitwidths:
      | blk = gcb;
      | mode = get_param(blk, 'mode');
      | current_widths = eval(get_param(blk, 'bitwidths'));
      | if (strcmp(mode, 'one value') || strcmp(mode, 'fields of equal size')) && (length(current_widths) > 1),
      |     error('Only one width may be specified for this mode.');
      | elseif strcmp(mode, 'fields of arbitrary size')
      |     current_names = textscan(strtrim(strrep(strrep(get_param(blk, 'names'), ']', ''), '[', '')), '%s');
      |     current_names = current_names{1};
      |     numios = length(current_names);
      |     if length(current_widths) ~= numios,
      |         error('%d field names specified, but %d widths?', numios, length(current_widths));
      |     end
      | end
      | total_width = 0;
      | for ctr = 1 : length(current_widths),
      |     total_width = total_width + current_widths(ctr);
      | end
      | if total_width > 32,
      |     error('Total width must be 32 or less, set to %d.', total_width);
      | end
      mask Callback arith_types:
      | blk = gcb;
      | mode = get_param(blk, 'mode');
      | current_types = eval(get_param(blk, 'arith_types'));
      | numios = length(current_types);
      | if (strcmp(mode, 'one value') || strcmp(mode, 'fields of equal size')) && (length(current_types) > 1),
      |     error('Only one type may be specified for this mode.');
      | elseif strcmp(mode, 'fields of arbitrary size')
      |     current_names = textscan(strtrim(strrep(strrep(get_param(blk, 'names'), ']', ''), '[', '')), '%s');
      |     current_names = current_names{1};
      |     numios = length(current_names);
      |     if length(current_types) ~= numios,
      |         error('%d field names specified, but %d types?', numios, length(current_types));
      |     end
      | end
      | problem = 0;
      | for ctr = 1 : numios,
      |     t = current_types(ctr);
      |     if (t < 0) || (t > 2),
      |         problem = t;
      |         ctr = numios + 1;
      |     end
      | end
      | if problem ~= 0,
      |     error('Type cannot be %i, must be 0, 1 or 2.', problem);
      | end
      mask Callback bin_pts:
      | blk = gcb;
      | mode = get_param(blk, 'mode');
      | current_bins = eval(get_param(blk, 'bin_pts'));
      | if (strcmp(mode, 'one value') || strcmp(mode, 'fields of equal size')) && (length(current_bins) > 1),
      |     error('Only one binary pt may be specified for this mode.');
      | elseif strcmp(mode, 'fields of arbitrary size')
      |     current_names = textscan(strtrim(strrep(strrep(get_param(blk, 'names'), ']', ''), '[', '')), '%s');
      |     current_names = current_names{1};
      |     numios = length(current_names);
      |     if length(current_bins) ~= numios,
      |         error('%d field names specified, but %d binary pts?', numios, length(current_bins));
      |     end
      | end
  vaccout3 : Subsystem  Tag=xps:sw_reg  AncestorBlock=xps_library/software register  mask(swreg){mode=fields of arbitrary size, io_dir=To Processor, io_delay=1, sample_period=1, names=[ready_cnt eof_cnt], bitwidths=[16 16], arith_types=[0 0], bin_pts=0, sim_port=off, show_format=off}
      mask prompts: io_dir "I/O direction"; io_delay "I/O delay"; sample_period "Sample period"; names "Names [msb ... lsb]:"; bitwidths "Bitwidths [msb ... lsb]:"; arith_types "Types (ufix=0, fix=1, bool=2) [msb ... lsb]:"; bin_pts "Binary pts [msb ... lsb]:"; sim_port "Provide sim input/output?"; show_format "Print format string?"
      mask init:
      | swreg_init(gcb)
      settings: AttributesFormatString=2 outputs
      mask TypeOptions mode: one value | fields of equal size | fields of arbitrary size
      mask Callback mode: swreg_cb(gcb);
      mask TypeOptions io_dir: To Processor | From Processor
      mask Callback io_dir:
      | mask_enables = get_param(gcb, 'MaskEnables');
      | mask_names = get_param(gcb, 'MaskNames');
      | if strcmp(get_param(gcb, 'io_dir'), 'To Processor'),
      |     mask_enables{ismember(mask_names, 'sample_period')} = 'off';
      | else
      |     mask_enables{ismember(mask_names, 'sample_period')} = 'on';
      | end
      | set_param(gcb, 'MaskEnables', mask_enables);
      mask Callback bitwidths:
      | blk = gcb;
      | mode = get_param(blk, 'mode');
      | current_widths = eval(get_param(blk, 'bitwidths'));
      | if (strcmp(mode, 'one value') || strcmp(mode, 'fields of equal size')) && (length(current_widths) > 1),
      |     error('Only one width may be specified for this mode.');
      | elseif strcmp(mode, 'fields of arbitrary size')
      |     current_names = textscan(strtrim(strrep(strrep(get_param(blk, 'names'), ']', ''), '[', '')), '%s');
      |     current_names = current_names{1};
      |     numios = length(current_names);
      |     if length(current_widths) ~= numios,
      |         error('%d field names specified, but %d widths?', numios, length(current_widths));
      |     end
      | end
      | total_width = 0;
      | for ctr = 1 : length(current_widths),
      |     total_width = total_width + current_widths(ctr);
      | end
      | if total_width > 32,
      |     error('Total width must be 32 or less, set to %d.', total_width);
      | end
      mask Callback arith_types:
      | blk = gcb;
      | mode = get_param(blk, 'mode');
      | current_types = eval(get_param(blk, 'arith_types'));
      | numios = length(current_types);
      | if (strcmp(mode, 'one value') || strcmp(mode, 'fields of equal size')) && (length(current_types) > 1),
      |     error('Only one type may be specified for this mode.');
      | elseif strcmp(mode, 'fields of arbitrary size')
      |     current_names = textscan(strtrim(strrep(strrep(get_param(blk, 'names'), ']', ''), '[', '')), '%s');
      |     current_names = current_names{1};
      |     numios = length(current_names);
      |     if length(current_types) ~= numios,
      |         error('%d field names specified, but %d types?', numios, length(current_types));
      |     end
      | end
      | problem = 0;
      | for ctr = 1 : numios,
      |     t = current_types(ctr);
      |     if (t < 0) || (t > 2),
      |         problem = t;
      |         ctr = numios + 1;
      |     end
      | end
      | if problem ~= 0,
      |     error('Type cannot be %i, must be 0, 1 or 2.', problem);
      | end
      mask Callback bin_pts:
      | blk = gcb;
      | mode = get_param(blk, 'mode');
      | current_bins = eval(get_param(blk, 'bin_pts'));
      | if (strcmp(mode, 'one value') || strcmp(mode, 'fields of equal size')) && (length(current_bins) > 1),
      |     error('Only one binary pt may be specified for this mode.');
      | elseif strcmp(mode, 'fields of arbitrary size')
      |     current_names = textscan(strtrim(strrep(strrep(get_param(blk, 'names'), ']', ''), '[', '')), '%s');
      |     current_names = current_names{1};
      |     numios = length(current_names);
      |     if length(current_bins) ~= numios,
      |         error('%d field names specified, but %d binary pts?', numios, length(current_bins));
      |     end
      | end
  tag scope: acc_len=global, bf0_id=global, bf0_n_partitions=global, bf0_partition_offset0=global, bf0_partition_offset1=global, bf0_partition_offset2=global, bf0_partition_offset3=global, bf0_rst=global, bf0_tx_pkt0=global, bf0_tx_pkt1=global, bf0_tx_pkt2=global, bf0_tx_pkt3=global, bf0_txen=global, bf1_id=global, bf1_n_partitions=global, bf1_partition_offset0=global, bf1_partition_offset1=global, bf1_partition_offset2=global, bf1_partition_offset3=global, bf1_rst=global, bf1_tx_pkt0=global, bf1_tx_pkt1=global, bf1_tx_pkt2=global, bf1_tx_pkt3=global, bf1_txen=global, bf_antenna=global, bf_beng=global, bf_data_id=global, bf_stream=global, bf_time_id=global, bf_valctrl_bw=global, bf_valctrl_dupl=global, bf_valctrl_filt=global, bf_valctrl_quant=global, bf_value_bw=global, bf_value_dupl=global, bf_value_filt=global, bf_value_quant=global, board_id=global, cnt_rst=global, err_calfail0=global, err_calfail1=global, err_calfail2=global, err_calfail3=global, err_input_of0=global, err_input_of1=global, err_input_of2=global, err_input_of3=global, err_output_of0=global, err_output_of1=global, err_output_of2=global, err_output_of3=global, err_parity0=global, err_parity1=global, err_parity2=global, err_parity3=global, err_rst0=global, err_rst1=global, err_rst2=global, err_rst3=global, flags0=global, flags1=global, flags2=global, flags3=global, flush0=global, flush1=global, gap_size0=global, gap_size1=global, gap_size2=global, gap_size3=global, gbe_rx_bad0=global, gbe_rx_bad1=global, gbe_rx_bad2=global, gbe_rx_bad3=global, gbe_txen=global, go0=global, go1=global, go2=global, go3=global, spead_data0=global, spead_data1=global, spead_data2=global, spead_data3=global, spead_eof0=global, spead_eof1=global, spead_eof2=global, spead_eof3=global, spead_error0=global, spead_error1=global, spead_error2=global, spead_error3=global, spead_hdr1_0=global, spead_hdr1_1=global, spead_hdr1_2=global, spead_hdr1_3=global, spead_hdr2_0=global, spead_hdr2_1=global, spead_hdr2_2=global, spead_hdr2_3=global, spead_hdr3_0=global, spead_hdr3_1=global, spead_hdr3_2=global, spead_hdr3_3=global, spead_hdr4_0=global, spead_hdr4_1=global, spead_hdr4_2=global, spead_hdr4_3=global, spead_valid0=global, spead_valid1=global, spead_valid2=global, spead_valid3=global, tvg_flags_sel0=global, tvg_flags_sel1=global, tvg_flags_sel2=global, tvg_flags_sel3=global, vacc_ld_arm=global, vacc_ld_immediate=global, vacc_ld_time=global, vacc_rst=global, vacc_tvg_sel=global, vaccin_newtvg=global, xeng_tvg_sel=global
  wires:
  master_reset_sim4/1 -> acc_len/1(sim_1)
  acc_len/1(in_reg) -> Delay21/1(d)
  [gbe_rxvld0] -> Delay6/1(d)
  [gbe_rxdata0] -> Delay2/1(d)
  [gbe_rxeof0] -> Delay7/1(d)
  gbe0/1(led_up) -> [gbe_up0]
  gbe0/2(led_rx) -> Terminator7/1
  gbe0/3(led_tx) -> Terminator13/1
  gbe0/4(tx_afull) -> Terminator14/1
  gbe0/5(tx_overflow) -> [gbe_tx_over0]
  gbe0/12(rx_overrun) -> Terminator36/1
  gbe0/11(rx_bad_frame) -> [gbe_rx_bad0]
  gbe0/6(rx_data) -> [gbe_rxdata0]
  gbe0/7(rx_valid) -> [gbe_rxvld0]
  gbe0/8(rx_source_ip) -> Terminator15/1
  gbe0/9(rx_source_port) -> Terminator35/1
  gbe0/10(rx_end_of_frame) -> [gbe_rxeof0]
  Constant2/1 -> gbe0/7(rx_ack)
  Constant8/1 -> gbe0/8(rx_overrun_ack)
  gbe_porttx/1(in_reg) -> Delay9/1(d)
  gbe_iptx/1(in_reg) -> Delay10/1(d)
  Delay9/1(q) -> [gbe_txport]
  Delay10/1(q) -> [gbe_txip]
  board_id/1(in_reg) -> Delay72/1(d)
  Constant9/1 -> gbe1/7(rx_ack)
  Constant13/1 -> gbe1/8(rx_overrun_ack)
  gbe1/11(rx_bad_frame) -> [gbe_rx_bad1]
  gbe1/5(tx_overflow) -> [gbe_tx_over1]
  gbe1/1(led_up) -> [gbe_up1]
  control/3(in_cnt_rst) -> pipeline3/1(d)
  control/1(in_vacc_rst) -> pipeline12/1(d)
  control/2(in_status_clr) -> pipeline1/1(d)
  pipeline8/1(q) -> [flasher_en]
  pipeline5/1(q) -> [gbe_txen]
  pipeline2/1(q) -> [gbe_rst]
  edge_detect/1(out) -> [cnt_rst]
  edge_detect3/1(out) -> [clr_status]
  edge_detect2/1(out) -> [vacc_rst]
  edge_detect1/1(out) -> [gbe_debug_rst]
  control/6(in_gbe_debug_rst) -> pipeline4/1(d)
  [gbe_debug_rst] -> gbe0/9(debug_rst)
  [gbe_debug_rst] -> gbe1/9(debug_rst)
  gbe1/2(led_rx) -> Terminator38/1
  gbe1/3(led_tx) -> Terminator50/1
  gbe1/4(tx_afull) -> Terminator51/1
  gbe1/8(rx_source_ip) -> Terminator52/1
  gbe1/9(rx_source_port) -> Terminator53/1
  gbe1/12(rx_overrun) -> Terminator54/1
  gbe1/6(rx_data) -> [gbe_rxdata1]
  gbe1/7(rx_valid) -> [gbe_rxvld1]
  gbe1/10(rx_end_of_frame) -> [gbe_rxeof1]
  Delay2/1(q) -> spead_unpack0/1(pkt_data)
  Delay6/1(q) -> spead_unpack0/2(pkt_valid)
  Delay7/1(q) -> spead_unpack0/3(pkt_eof)
  spead_unpack0/1(pkt_start) -> Terminator28/1
  spead_unpack0/2(data64) -> [spead_data0]
  spead_unpack0/3(valid64) -> [spead_valid0]
  spead_unpack0/4(eof64) -> [spead_eof0]
  spead_unpack0/5(error) -> [spead_error0]
  spead_unpack0/6(hdr_heap_id) -> Terminator2/1
  spead_unpack0/7(hdr_heap_size) -> Terminator3/1
  spead_unpack0/8(hdr_heap_offset) -> Terminator4/1
  spead_unpack0/9(hdr_pkt_len) -> Terminator5/1
  spead_unpack0/11(hdr6_0x4101_DIR) -> [spead_hdr2_0]
  spead_unpack0/12(hdr7_0x4102_DIR) -> [spead_hdr3_0]
  spead_unpack0/13(hdr8_0x4103_DIR) -> [spead_hdr4_0]
  spead_unpack0/14(hdr9_0x4300) -> Terminator31/1
  Delay72/1(q) -> [board_id]
  [gbe_rxvld1] -> Delay29/1(d)
  [gbe_rxdata1] -> Delay17/1(d)
  [gbe_rxeof1] -> Delay34/1(d)
  Delay17/1(q) -> spead_unpack1/1(pkt_data)
  Delay29/1(q) -> spead_unpack1/2(pkt_valid)
  Delay34/1(q) -> spead_unpack1/3(pkt_eof)
  spead_unpack1/1(pkt_start) -> Terminator23/1
  spead_unpack1/2(data64) -> [spead_data1]
  spead_unpack1/3(valid64) -> [spead_valid1]
  spead_unpack1/4(eof64) -> [spead_eof1]
  spead_unpack1/5(error) -> [spead_error1]
  spead_unpack1/6(hdr_heap_id) -> Terminator17/1
  spead_unpack1/7(hdr_heap_size) -> Terminator18/1
  spead_unpack1/8(hdr_heap_offset) -> Terminator19/1
  spead_unpack1/9(hdr_pkt_len) -> Terminator11/1
  spead_unpack1/11(hdr6_0x4101_DIR) -> [spead_hdr2_1]
  spead_unpack1/12(hdr7_0x4102_DIR) -> [spead_hdr3_1]
  spead_unpack1/13(hdr8_0x4103_DIR) -> [spead_hdr4_1]
  spead_unpack1/14(hdr9_0x4300) -> Terminator32/1
  edge_detect5/1(out) -> [reord_snaptrig]
  pipeline13/1(q) -> [reord_snaptrigsel]
  control/8(in_reord_snaptrig) -> pipeline6/1(d)
  tvg_control/1(in_xeng) -> pipeline7/1(d)
  pipeline7/1(q) -> [xeng_tvg_sel]
  pipeline11/1(q) -> [vacc_tvg_sel]
  tvg_control/2(in_vacc) -> pipeline11/1(d)
  vacc_time_msw/3(in_msw) -> Delay19/1(d)
  vacc_time_msw/1(in_arm) -> Delay16/1(d)
  Concat10/1 -> [vacc_ld_time]
  vacc_time_msw/2(in_immediate) -> Delay18/1(d)
  vacc_time_lsw/1(in_lsw) -> Delay20/1(d)
  spead_unpack0/10(hdr5_0x1600_DIR) -> [spead_hdr1_0]
  spead_unpack1/10(hdr5_0x1600_DIR) -> [spead_hdr1_1]
  vaccin_newtvg/1(in_reg) -> pipeline9/1(d)
  Delay16/1(q) -> [vacc_ld_arm]
  Delay18/1(q) -> [vacc_ld_immediate]
  Delay19/1(q) -> Concat10/1
  Delay20/1(q) -> Concat10/2
  Delay21/1(q) -> [acc_len]
  pipeline9/1(q) -> [vaccin_newtvg]
  flags0/2(in_flags) -> pipeline16/1(d)
  flags0/1(in_tvg_en) -> pipeline15/1(d)
  flags1/1(in_tvg_en) -> pipeline17/1(d)
  pipeline15/1(q) -> [tvg_flags_sel0]
  pipeline16/1(q) -> [flags0]
  pipeline18/1(q) -> [flags1]
  pipeline17/1(q) -> [tvg_flags_sel1]
  pipeline20/1(q) -> [flags2]
  pipeline22/1(q) -> [flags3]
  pipeline19/1(q) -> [tvg_flags_sel2]
  pipeline21/1(q) -> [tvg_flags_sel3]
  [gbe_rst] -> gbe0/1(rst)
  [gbe_txd0] -> gbe0/2(tx_data)
  [gbe_txvld0] -> gbe0/3(tx_valid)
  [gbe_txip] -> gbe0/4(tx_dest_ip)
  [gbe_txport] -> gbe0/5(tx_dest_port)
  [gbe_txeof0] -> gbe0/6(tx_end_of_frame)
  [gbe_rst] -> gbe1/1(rst)
  [gbe_txd1] -> gbe1/2(tx_data)
  [gbe_txvld1] -> gbe1/3(tx_valid)
  [gbe_txip] -> gbe1/4(tx_dest_ip)
  [gbe_txport] -> gbe1/5(tx_dest_port)
  [gbe_txeof1] -> gbe1/6(tx_end_of_frame)
  miss_cnt2/1(spectr_cnt) -> reordcnt_spec2/1(out_reg)
  miss_cnt2/3(recv_ctr) -> reordcnt_recv2/1(out_reg)
  miss_cnt2/5(timeout_errctr) -> reorderr_timeout2/1(out_reg)
  miss_cnt2/2(last_missed_ant) -> reord_missant2/1(out_reg)
  miss_cnt2/4(recv_errctr) -> reorderr_recv2/1(out_reg)
  miss_cnt2/6(pktdisc_errctr) -> reorderr_disc2/1(out_reg)
  [cnt_rst] -> vacc_monitor4/1(cnt_rst), vacc_monitor6/1(cnt_rst)
  vacc_monitor6/5(parity_cnt) -> vacc_errors2/5(out_parity)
  vacc_monitor6/3(rst_cnt) -> vacc_errors2/3(out_rst)
  vacc_monitor6/4(outof_cnt) -> vacc_errors2/4(out_outputof)
  vacc_monitor6/2(inof_cnt) -> vacc_errors2/2(out_inputof)
  vacc_monitor6/1(cal_cnt) -> vacc_errors2/1(out_calfail)
  [err_parity2] -> vacc_monitor6/6(parity)
  [err_rst2] -> vacc_monitor6/4(rst)
  [err_calfail2] -> vacc_monitor6/2(cal)
  [err_input_of2] -> vacc_monitor6/3(inof)
  [err_output_of2] -> vacc_monitor6/5(outof)
  [vacc_ld_stat2] -> Delay39/1(d)
  vacc_monitor5/1(pkt_cnt) -> packcnt_out2/1(out_reg)
  vacc_monitor5/2(error_cnt) -> packerr_2/1(out_reg)
  [cnt_rst] -> vacc_monitor5/1(cnt_rst)
  [pack_txeof2] -> vacc_monitor5/2(eof)
  [pack_err2] -> vacc_monitor5/3(error)
  [cnt_rst] -> Subsystem5/1(rst)
  [spead_valid0] -> Subsystem5/2(we)
  [spead_eof0] -> Subsystem5/3(eof)
  [spead_error0] -> Subsystem5/4(flag)
  Subsystem5/1(rx_cnt) -> rx_cnt0/1(out_reg)
  Subsystem5/2(err_cnt) -> rx_err_cnt0/1(out_reg)
  spead_time_check/1(lsbzero0) -> speadtime_lsbzero/1(out_spead0)
  spead_time_check/2(lsbzero1) -> speadtime_lsbzero/2(out_spead1)
  [cnt_rst] -> Subsystem2/1(rst)
  pipeline24/1(q) -> [gap_size3]
  pipeline23/1(q) -> [gap_size2]
  pipeline14/1(q) -> [gap_size1]
  pipeline10/1(q) -> [gap_size0]
  flags1/2(in_flags) -> pipeline18/1(d)
  flags2/1(in_tvg_en) -> pipeline19/1(d)
  flags2/2(in_flags) -> pipeline20/1(d)
  flags3/1(in_tvg_en) -> pipeline21/1(d)
  flags3/2(in_flags) -> pipeline22/1(d)
  pipeline12/1(q) -> edge_detect2/1(in)
  pipeline1/1(q) -> edge_detect3/1(in)
  pipeline3/1(q) -> edge_detect/1(in)
  control/4(in_gbe_rst) -> pipeline2/1(d)
  pipeline4/1(q) -> edge_detect1/1(in)
  pipeline6/1(q) -> edge_detect5/1(in)
  control/5(in_gbe_txen) -> pipeline5/1(d)
  control/7(in_flasher_en) -> pipeline8/1(d)
  control/9(in_reord_snaptrigsel) -> pipeline13/1(d)
  control/10(in_unpack_snapwesel) -> pipeline25/1(d)
  pipeline25/1(q) -> [unpack_snapwesel]
  [vacc_err_flags2] -> bus_expand9/1(bus_in)
  [gbe_up1] -> Inverter4/1
  [clr_status] -> latch2/1(reset)
  [pack_err2] -> latch2/15(pack_err)
  [pre_rx_dest_err2] -> latch2/3(rx_dest_err)
  [pre_feng_rx_err2] -> latch2/4(feng_rx_err)
  [pre_ndiode_en2] -> latch2/9(noise_diode_en)
  [pre_adc_err2] -> latch2/8(adc_over)
  [vacc_err2] -> latch2/10(vacc_err)
  [pre_spead_err2] -> latch2/11(rx_bad_pkt)
  [pre_feng_chk_err2] -> latch2/7(feng_chk_err)
  [gbe_rx_bad1] -> latch2/12(rx_bad_frame)
  [pre_feng_qdr_err2] -> latch2/6(feng_qdr_err)
  [gbe_tx_over1] -> latch2/13(tx_over)
  [pre_fft_err2] -> latch2/5(fft_err)
  [reord_recverr2] -> latch2/14(xeng_bad_dat)
  Inverter4/1 -> latch2/2(gbe_down)
  Inverter3/1 -> latch2/16(rx)
  [accumulating2] -> latch2/17(tx)
  [reord_recverr2] -> Inverter3/1
  miss_cnt1/1(spectr_cnt) -> reordcnt_spec1/1(out_reg)
  miss_cnt1/2(last_missed_ant) -> reord_missant1/1(out_reg)
  miss_cnt1/3(recv_ctr) -> reordcnt_recv1/1(out_reg)
  miss_cnt1/4(recv_errctr) -> reorderr_recv1/1(out_reg)
  miss_cnt1/5(timeout_errctr) -> reorderr_timeout1/1(out_reg)
  miss_cnt1/6(pktdisc_errctr) -> reorderr_disc1/1(out_reg)
  bus_expand6/1(msb_out2) -> vacc_ld_status1/1(out_armcnt)
  bus_expand6/2(lsb_out1) -> vacc_ld_status1/2(out_ldcnt)
  vacc_monitor9/5(parity_cnt) -> vacc_errors1/5(out_parity)
  vacc_monitor9/3(rst_cnt) -> vacc_errors1/3(out_rst)
  vacc_monitor9/4(outof_cnt) -> vacc_errors1/4(out_outputof)
  vacc_monitor9/2(inof_cnt) -> vacc_errors1/2(out_inputof)
  vacc_monitor9/1(cal_cnt) -> vacc_errors1/1(out_calfail)
  Delay8/1(q) -> bus_expand6/1(bus_in)
  [vacc_ld_stat1] -> Delay8/1(d)
  [err_parity1] -> vacc_monitor9/6(parity)
  [err_rst1] -> vacc_monitor9/4(rst)
  [err_calfail1] -> vacc_monitor9/2(cal)
  [err_input_of1] -> vacc_monitor9/3(inof)
  [err_output_of1] -> vacc_monitor9/5(outof)
  [vacc_err_flags1] -> bus_expand1/1(bus_in)
  vacc_monitor2/1(pkt_cnt) -> packcnt_out1/1(out_reg)
  vacc_monitor2/2(error_cnt) -> packerr_1/1(out_reg)
  [cnt_rst] -> vacc_monitor2/1(cnt_rst)
  [pack_txeof1] -> vacc_monitor2/2(eof)
  [pack_err1] -> vacc_monitor2/3(error)
  [gbe_up0] -> Inverter2/1
  [clr_status] -> latch1/1(reset)
  [pack_err1] -> latch1/15(pack_err)
  [pre_rx_dest_err1] -> latch1/3(rx_dest_err)
  [pre_feng_rx_err1] -> latch1/4(feng_rx_err)
  [pre_ndiode_en1] -> latch1/9(noise_diode_en)
  [pre_adc_err1] -> latch1/8(adc_over)
  [vacc_err1] -> latch1/10(vacc_err)
  [pre_spead_err1] -> latch1/11(rx_bad_pkt)
  [pre_feng_chk_err1] -> latch1/7(feng_chk_err)
  [gbe_rx_bad0] -> latch1/12(rx_bad_frame)
  [pre_feng_qdr_err1] -> latch1/6(feng_qdr_err)
  [gbe_tx_over0] -> latch1/13(tx_over)
  [pre_fft_err1] -> latch1/5(fft_err)
  [reord_recverr1] -> latch1/14(xeng_bad_dat)
  Inverter2/1 -> latch1/2(gbe_down)
  Inverter1/1 -> latch1/16(rx)
  [accumulating1] -> latch1/17(tx)
  [reord_recverr1] -> Inverter1/1
  miss_cnt0/3(recv_ctr) -> reordcnt_recv0/1(out_reg)
  miss_cnt0/1(spectr_cnt) -> reordcnt_spec0/1(out_reg)
  miss_cnt0/2(last_missed_ant) -> reord_missant0/1(out_reg)
  miss_cnt0/4(recv_errctr) -> reorderr_recv0/1(out_reg)
  miss_cnt0/5(timeout_errctr) -> reorderr_timeout0/1(out_reg)
  miss_cnt0/6(pktdisc_errctr) -> reorderr_disc0/1(out_reg)
  [vacc_newacc0] -> vacc_monitor1/2(new_acc)
  [vacc_err0] -> vacc_monitor1/5(error)
  [cnt_rst] -> vacc_monitor1/1(cnt_rst), vacc_monitor8/1(cnt_rst)
  [vacc_ld_stat0] -> Delay4/1(d)
  bus_expand5/1(msb_out2) -> vacc_ld_status0/1(out_armcnt)
  bus_expand5/2(lsb_out1) -> vacc_ld_status0/2(out_ldcnt)
  vacc_monitor8/5(parity_cnt) -> vacc_errors0/5(out_parity)
  vacc_monitor8/3(rst_cnt) -> vacc_errors0/3(out_rst)
  vacc_monitor8/4(outof_cnt) -> vacc_errors0/4(out_outputof)
  vacc_monitor8/2(inof_cnt) -> vacc_errors0/2(out_inputof)
  vacc_monitor8/1(cal_cnt) -> vacc_errors0/1(out_calfail)
  [err_output_of0] -> vacc_monitor8/5(outof)
  [err_parity0] -> vacc_monitor8/6(parity)
  [err_rst0] -> vacc_monitor8/4(rst)
  [err_input_of0] -> vacc_monitor8/3(inof)
  [err_calfail0] -> vacc_monitor8/2(cal)
  [vacc_err_flags0] -> bus_expand2/1(bus_in)
  vacc_monitor3/1(pkt_cnt) -> packcnt_out0/1(out_reg)
  vacc_monitor3/2(error_cnt) -> packerr_0/1(out_reg)
  [pack_txeof0] -> vacc_monitor3/2(eof)
  [pack_err0] -> vacc_monitor3/3(error)
  [cnt_rst] -> vacc_monitor3/1(cnt_rst)
  latch0/3(feng_rx_err_reg) -> status0/3(out_feng_rx_err)
  latch0/2(rx_dest_err_reg) -> status0/2(out_rx_dest_err)
  latch0/1(gbe_down_reg) -> status0/1(out_gbe_down)
  latch0/16(tx_reg) -> status0/16(out_txing_data)
  latch0/15(rx_reg) -> status0/15(out_rxing_data)
  latch0/12(tx_over_reg) -> status0/12(out_tx_over)
  latch0/6(feng_chk_err_reg) -> status0/6(out_feng_chk_err)
  latch0/14(pack_err_reg) -> status0/14(out_pack_err)
  latch0/10(rx_bad_pkt_reg) -> status0/10(out_rx_bad_pkt)
  latch0/7(adc_over_reg) -> status0/7(out_adc_over)
  latch0/9(vacc_err_reg) -> status0/9(out_vacc_err)
  latch0/4(fft_err_reg) -> status0/4(out_fft_err)
  latch0/11(rx_bad_frame_reg) -> status0/11(out_rx_bad_frame)
  latch0/5(feng_qdr_err_reg) -> status0/5(out_feng_qdr_err)
  latch0/8(noise_diode_en_reg) -> status0/8(out_noise_diode_en)
  latch0/13(xeng_bad_dat_reg) -> status0/13(out_xeng_bad_dat)
  latch0/17(data_bad) -> [data_in_bad0]
  latch0/18(error) -> [err0]
  [gbe_up0] -> Inverter5/1
  [clr_status] -> latch0/1(reset)
  [pack_err0] -> latch0/15(pack_err)
  [pre_rx_dest_err0] -> latch0/3(rx_dest_err)
  [pre_feng_rx_err0] -> latch0/4(feng_rx_err)
  [pre_ndiode_en0] -> latch0/9(noise_diode_en)
  [pre_adc_err0] -> latch0/8(adc_over)
  [vacc_err0] -> latch0/10(vacc_err)
  [pre_spead_err0] -> latch0/11(rx_bad_pkt)
  [pre_feng_chk_err0] -> latch0/7(feng_chk_err)
  [gbe_rx_bad0] -> latch0/12(rx_bad_frame)
  [pre_feng_qdr_err0] -> latch0/6(feng_qdr_err)
  [gbe_tx_over0] -> latch0/13(tx_over)
  [pre_fft_err0] -> latch0/5(fft_err)
  [reord_recverr0] -> latch0/14(xeng_bad_dat)
  Inverter5/1 -> latch0/2(gbe_down)
  Inverter/1 -> latch0/16(rx)
  [accumulating0] -> latch0/17(tx)
  [reord_recverr0] -> Inverter/1
  [gbe_up1] -> Inverter7/1
  [clr_status] -> latch3/1(reset)
  [pack_err3] -> latch3/15(pack_err)
  [pre_rx_dest_err3] -> latch3/3(rx_dest_err)
  [pre_feng_rx_err3] -> latch3/4(feng_rx_err)
  [pre_ndiode_en3] -> latch3/9(noise_diode_en)
  [pre_adc_err3] -> latch3/8(adc_over)
  [vacc_err3] -> latch3/10(vacc_err)
  [pre_spead_err3] -> latch3/11(rx_bad_pkt)
  [pre_feng_chk_err3] -> latch3/7(feng_chk_err)
  [gbe_rx_bad1] -> latch3/12(rx_bad_frame)
  [pre_feng_qdr_err3] -> latch3/6(feng_qdr_err)
  [gbe_tx_over1] -> latch3/13(tx_over)
  [pre_fft_err3] -> latch3/5(fft_err)
  [reord_recverr3] -> latch3/14(xeng_bad_dat)
  Inverter7/1 -> latch3/2(gbe_down)
  Inverter6/1 -> latch3/16(rx)
  [accumulating3] -> latch3/17(tx)
  [reord_recverr3] -> Inverter6/1
  vacc_monitor7/1(pkt_cnt) -> packcnt_out3/1(out_reg)
  vacc_monitor7/2(error_cnt) -> packerr_3/1(out_reg)
  [cnt_rst] -> vacc_monitor7/1(cnt_rst)
  [pack_txeof3] -> vacc_monitor7/2(eof)
  [pack_err3] -> vacc_monitor7/3(error)
  [vacc_ld_stat3] -> Delay5/1(d)
  [err_output_of3] -> vacc_monitor11/5(outof)
  [err_parity3] -> vacc_monitor11/6(parity)
  [err_rst3] -> vacc_monitor11/4(rst)
  [err_input_of3] -> vacc_monitor11/3(inof)
  [err_calfail3] -> vacc_monitor11/2(cal)
  vacc_monitor11/1(cal_cnt) -> vacc_errors3/1(out_calfail)
  vacc_monitor11/2(inof_cnt) -> vacc_errors3/2(out_inputof)
  vacc_monitor11/3(rst_cnt) -> vacc_errors3/3(out_rst)
  vacc_monitor11/4(outof_cnt) -> vacc_errors3/4(out_outputof)
  vacc_monitor11/5(parity_cnt) -> vacc_errors3/5(out_parity)
  [vacc_err_flags3] -> bus_expand4/1(bus_in)
  miss_cnt3/3(recv_ctr) -> reordcnt_recv3/1(out_reg)
  miss_cnt3/1(spectr_cnt) -> reordcnt_spec3/1(out_reg)
  miss_cnt3/2(last_missed_ant) -> reord_missant3/1(out_reg)
  miss_cnt3/4(recv_errctr) -> reorderr_recv3/1(out_reg)
  miss_cnt3/5(timeout_errctr) -> reorderr_timeout3/1(out_reg)
  miss_cnt3/6(pktdisc_errctr) -> reorderr_disc3/1(out_reg)
  [error0] -> Logical/1
  [error1] -> Logical/2
  [error2] -> Logical/3
  [error3] -> Logical/4
  [warning0] -> Logical1/1
  [warning1] -> Logical1/2
  [warning2] -> Logical1/3
  [warning3] -> Logical1/4
  Logical/1 -> Slice/1
  Logical1/1 -> Slice1/1
  [cnt_rst] -> Delay3/2, Delay/2
  Delay/1 -> status/1(out_error)
  Delay3/1 -> status/2(out_warning)
  Slice/1 -> Delay/3, Delay/1
  Slice1/1 -> Delay3/3, Delay3/1
  Delay4/1(q) -> bus_expand5/1(bus_in)
  gap_size/1(in_gap_size) -> Relational/2, Delay1/1
  Delay1/1 -> Register/1, Relational/1
  Relational/1 -> Register/2
  Register/1 -> pipeline24/1(d), pipeline23/1(d), pipeline14/1(d), pipeline10/1(d)
  Delay5/1(q) -> bus_expand8/1(bus_in)
  [pack_ready0] -> vacc_monitor1/3(ready)
  [pack_txeof0] -> vacc_monitor1/4(eof)
  vacc_monitor1/2(ready_cnt) -> vaccout0/1(out_ready_cnt)
  vacc_monitor1/1(acc_cnt) -> vacccnt0/1(out_reg)
  vacc_monitor1/4(error_cnt) -> vaccerr0/1(out_reg)
  vacc_monitor1/3(eof_cnt) -> vaccout0/2(out_eof_cnt)
  vacc_monitor10/2(ready_cnt) -> vaccout1/1(out_ready_cnt)
  vacc_monitor10/1(acc_cnt) -> vacccnt1/1(out_reg)
  vacc_monitor10/4(error_cnt) -> vaccerr1/1(out_reg)
  vacc_monitor10/3(eof_cnt) -> vaccout1/2(out_eof_cnt)
  [vacc_err1] -> vacc_monitor10/5(error)
  [pack_txeof1] -> vacc_monitor10/4(eof)
  [pack_ready1] -> vacc_monitor10/3(ready)
  [vacc_newacc1] -> vacc_monitor10/2(new_acc)
  [cnt_rst] -> vacc_monitor10/1(cnt_rst), vacc_monitor9/1(cnt_rst)
  bus_expand7/1(msb_out2) -> vacc_ld_status2/1(out_armcnt)
  bus_expand7/2(lsb_out1) -> vacc_ld_status2/2(out_ldcnt)
  vacc_monitor4/1(acc_cnt) -> vacccnt2/1(out_reg)
  Delay39/1(q) -> bus_expand7/1(bus_in)
  [vacc_err2] -> vacc_monitor4/5(error)
  [pack_ready2] -> vacc_monitor4/3(ready)
  [pack_txeof2] -> vacc_monitor4/4(eof)
  [vacc_newacc2] -> vacc_monitor4/2(new_acc)
  bus_expand8/1(msb_out2) -> vacc_ld_status3/1(out_armcnt)
  bus_expand8/2(lsb_out1) -> vacc_ld_status3/2(out_ldcnt)
  vacc_monitor12/2(ready_cnt) -> vaccout3/1(out_ready_cnt)
  vacc_monitor12/1(acc_cnt) -> vacccnt3/1(out_reg)
  vacc_monitor12/4(error_cnt) -> vaccerr3/1(out_reg)
  vacc_monitor12/3(eof_cnt) -> vaccout3/2(out_eof_cnt)
  [pack_ready2] -> vacc_monitor12/3(ready)
  [pack_txeof2] -> vacc_monitor12/4(eof)
  [vacc_err3] -> vacc_monitor12/5(error)
  [cnt_rst] -> vacc_monitor12/1(cnt_rst), vacc_monitor11/1(cnt_rst)
  [vacc_newacc3] -> vacc_monitor12/2(new_acc)
  vacc_monitor4/4(error_cnt) -> vaccerr2/1(out_reg)
  vacc_monitor4/3(eof_cnt) -> vaccout2/2(out_eof_cnt)
  vacc_monitor4/2(ready_cnt) -> vaccout2/1(out_ready_cnt)
  [flush0] -> latch0/18(flush)
  latch0/19(flush_reg) -> status0/17(out_flushed)
  [flush0] -> latch1/18(flush)
  latch1/15(rx_reg) -> status1/15(out_rxing_data)
  latch1/6(feng_chk_err_reg) -> status1/6(out_feng_chk_err)
  latch1/1(gbe_down_reg) -> status1/1(out_gbe_down)
  latch1/12(tx_over_reg) -> status1/12(out_tx_over)
  latch1/13(xeng_bad_dat_reg) -> status1/13(out_xeng_bad_dat)
  latch1/10(rx_bad_pkt_reg) -> status1/10(out_rx_bad_pkt)
  latch1/9(vacc_err_reg) -> status1/9(out_vacc_err)
  latch1/2(rx_dest_err_reg) -> status1/2(out_rx_dest_err)
  latch1/3(feng_rx_err_reg) -> status1/3(out_feng_rx_err)
  latch1/11(rx_bad_frame_reg) -> status1/11(out_rx_bad_frame)
  latch1/7(adc_over_reg) -> status1/7(out_adc_over)
  latch1/5(feng_qdr_err_reg) -> status1/5(out_feng_qdr_err)
  latch1/14(pack_err_reg) -> status1/14(out_pack_err)
  latch1/16(tx_reg) -> status1/16(out_txing_data)
  latch1/8(noise_diode_en_reg) -> status1/8(out_noise_diode_en)
  latch1/4(fft_err_reg) -> status1/4(out_fft_err)
  latch1/17(data_bad) -> [data_in_bad1]
  latch1/18(error) -> [err1]
  latch1/19(flush_reg) -> status1/17(out_flushed)
  [flush1] -> latch2/18(flush)
  [flush1] -> latch3/18(flush)
  latch2/14(pack_err_reg) -> status2/14(out_pack_err)
